simulink model "OffRoadMultibodyStage1_TireDamping_Cz20_20261101"  (R2026a)
settings: Solver=ode15s  StopTime=100  RelTol=2e-3  EnableMultiTasking=on
values from neighbouring files (symbols this model uses):
  goalX = goalPoseWorkflow(1)    [buildCustomPhysicalScenarioModel.m]    (also in correctCustomObstacle3Spawn.m; createScenarioIntegrationTestModel.m = goalPose(1); planAroundConfiguredObstacle.m = originalPath(end,1); restoreRoughTerrainWorkspace.m = goalXY(1))
  goalY = goalPoseWorkflow(2)    [buildCustomPhysicalScenarioModel.m]    (also in correctCustomObstacle3Spawn.m; createScenarioIntegrationTestModel.m = goalPose(2); planAroundConfiguredObstacle.m = originalPath(end,2); restoreRoughTerrainWorkspace.m = goalXY(2))
  obstacle3X = obs(3).centerXY(1)    [buildCustomPhysicalScenarioModel.m]    (also in correctCustomObstacle3Spawn.m = o3.centerXY(1); createScenarioIntegrationTestModel.m = obstacleXs(3); restoreRoughTerrainWorkspace.m = obstacleXs(3); runCustomObstacle5DelayedAblation32s.m = double(obs(3).centerXY(1)))
  obstacle3Y = obs(3).centerXY(2)    [buildCustomPhysicalScenarioModel.m]    (also in correctCustomObstacle3Spawn.m = o3.centerXY(2); createScenarioIntegrationTestModel.m = obstacleYs(3); restoreRoughTerrainWorkspace.m = obstacleYs(3); runCustomObstacle5DelayedAblation32s.m = double(obs(3).centerXY(2)))
  obstacleSpawnTime = [obstacleSpawnTime nan(1,4)]    [buildCustomPhysicalScenarioModel.m]    (also in correctCustomObstacle3Spawn.m = [[obs.spawnTime] nan(1,4)]; createScenarioIntegrationTestModel.m = [obs.spawnTime]; restoreRoughTerrainWorkspace.m = [obs.spawnTime]; runCustomObstacle5DelayedAblation32s.m = [[obs.spawnTime] nan(1,4)])
  obstacleXs = [obstacleXs nan(1,4)]    [buildCustomPhysicalScenarioModel.m]    (also in correctCustomObstacle3Spawn.m = [allCenters(:,1).' nan(1,4)]; createScenarioIntegrationTestModel.m = allCenters(:,1).'; onlineReplanFromPose.m = obstacleXs(valid); onlineReplanFromPoseGeometryAware.m = obstacleXs(valid))
  obstacleYs = [obstacleYs nan(1,4)]    [buildCustomPhysicalScenarioModel.m]    (also in correctCustomObstacle3Spawn.m = [allCenters(:,2).' nan(1,4)]; createScenarioIntegrationTestModel.m = allCenters(:,2).'; onlineReplanFromPose.m = obstacleYs(valid); onlineReplanFromPoseGeometryAware.m = obstacleYs(valid))
  originalPathPadded = [ ... (first row only)    [planAroundConfiguredObstacle.m]
  s = blockNames{k}    [inspectPhysicalScenarioModel.m]    (also in inspectSteeringControllerAndTransferFcn.m = strtrim(s); inspectSteeringJointSignalPath.m = valueToText(v); runCustomSolverProfiler40s.m = profileResult.summary)
  X = X(:)'    [launchElevationTerrainRoverViewer.m]    (also in launchElevationTerrainRoverViewerMultiDynamic.m; launchRoughTerrainScenarioEditor.m = double(evalin('base', 'X')); previewGeometryAwareObstaclePlanner.m = evalin('base','X'))
  Y = Y(:)    [launchElevationTerrainRoverViewer.m]    (also in launchElevationTerrainRoverViewerMultiDynamic.m; launchRoughTerrainScenarioEditor.m = double(evalin('base', 'Y')); previewGeometryAwareObstaclePlanner.m = evalin('base','Y'))
  Z = double(Z_multibody)    [inspectFailureLocation.m]    (also in launchElevationTerrainRoverViewer.m = ZGridSurface.'; launchElevationTerrainRoverViewerMultiDynamic.m = ZGridSurface.'; previewGeometryAwareObstaclePlanner.m = evalin('base','Z'))
libraries: nesl_utility x71, sm_lib x45, slpidlib x1
(part 1 of 2)
settings Model: Creator=sagar  LastModifiedBy=sagar
settings DebuggingCC: SubsystemReferenceDiagnosticForUnitTest=warning
settings SimscapeCC: SimscapeNominalValues="[{\"value\":\"1\",\"unit\":\"A\"},{\"value\":\"1\",\"unit\":\"bar\"},{\"value\":\"1\",\"unit\":\"cm^2\"},{\"value\":\"1\",\"unit\":\"cm^3/s\"},{\"value\":\"1\",\"unit\":\"kJ/kg\"},{\"value\":\"1\",\"unit\":\"kW\"},{\"value\":\"1\",\"unit\":\"l\"},{\"value\":\"1\",\"unit\":\"N\"},{\"value\":\"1\",\"unit\":\"N*m\"},{\"value\":\"1\",\"unit\":\"V\"}]"
settings ExplorerConfigSet: InternalSimMechanicsExplorerSettings=|
  | <ExplorerConfiguration>
  | 
  |   <canonicalview>default</canonicalview>
  | 
  |   <TilePanel>
  |     <TileInfo>
  |       <Tiles Columns="1" Count="1" Height="825" Rows="1" Width="1462">
  |         <Row Weight="1"/>
  |         <Column Weight="1"/>
  |         <Tile Height="1" Width="1" X="0" Y="0"/>
  |       </Tiles>
  |     </TileInfo>
  |     <SceneInfo>
  |       <SceneViewer>
  |         <IsThisViewStd>
  |           <IsStandardView>off</IsStandardView>
  |           <StandardViewName>Front</StandardViewName>
  |         </IsThisViewStd>
  |         <BGColor>
  |           <R>1</R>
  |           <G>1</G>
  |           <B>1</B>
  |           <A>1</A>
  |         </BGColor>
  |         <Camera>
  |           <DoPerspective>off</DoPerspective>
  |           <Position>
  |             <X>25</X>
  |             <Y>-125.54576462577884</Y>
  |             <Z>151.6388221817023</Z>
  |           </Position>
  |           <Center>
  |             <X>25</X>
  |             <Y>25</Y>
  |             <Z>1.0930575559234619</Z>
  |           </Center>
  |           <Up>
  |             <X>0</X>
  |             <Y>0.70710678118654757</Y>
  |             <Z>0.70710678118654757</Z>
  |           </Up>
  |           <XLim>20.406588216402103</XLim>
  |           <YLim>20.406588216402103</YLim>
  |           <ViewLimDist>0.01</ViewLimDist>
  |         </Camera>
  |       </SceneViewer>
  |     </SceneInfo>
  |   </TilePanel>
  | 
  |   <MechEditorPanel>
  |     <GfxPanelCameraMap/>
  |     <Cameras/>
  |     <VideoCreator>
  |       <IncludeTiles>All</IncludeTiles>
  |       <IncludeTime>on</IncludeTime>
  |       <IncludeWorldFrame>off</IncludeWorldFrame>
  |       <PlaybackSpeedRatio>1</PlaybackSpeedRatio>
  |       <FrameRate>30</FrameRate>
  |       <FrameSize>auto</FrameSize>
  |       <VideoFormat>UncompressedAVI</VideoFormat>
  |     </VideoCreator>
  |   </MechEditorPanel>
  | 
  |   <PlaybackSettings>
  |     <PlaybackSpeedFactor>16</PlaybackSpeedFactor>
  |   </PlaybackSettings>
  | 
  | </ExplorerConfiguration>

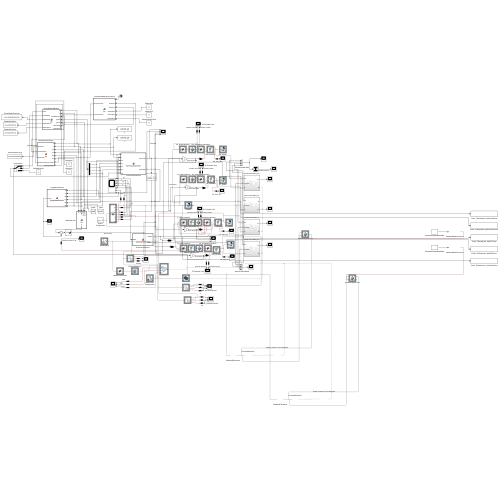
[thumbnail: Simulink's stored preview of the top-level diagram]
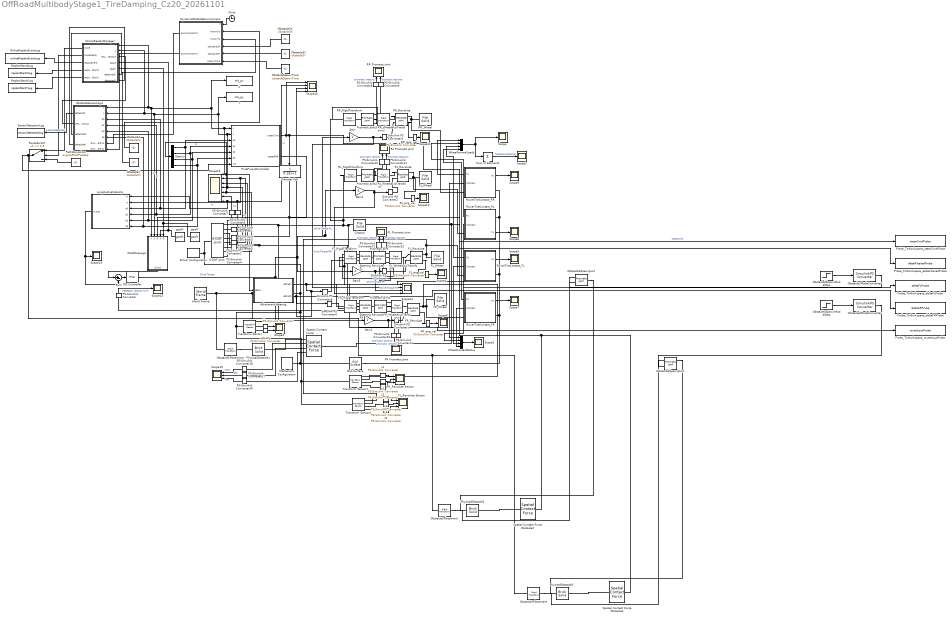
== system OffRoadMultibodyStage1_TireDamping_Cz20_20261101 ==
  6-DOF Joint : sm_lib/Joints/6-DOF Joint  JointMode=Normal  CompositeWrenchDir=FollowerOnBase  CompositeWrenchFrame=BaseFrame  SenseConstraintForce=off  SenseConstraintTorque=off  SenseTotalForce=off  SenseTotalTorque=off  PxPositionTargetSpecify=on  PxPositionTargetPriority=High  PxPositionTargetValue=4.53703703703703  PxPositionTargetValueUnits=m  PxVelocityTargetSpecify=off  PxVelocityTargetPriority=High  PxVelocityTargetValue=0  PxVelocityTargetValueUnits=m/s  PxEquilibriumPosition=0  PxEquilibriumPositionUnits=m  PxSpringStiffness=0  PxSpringStiffnessUnits=N/m  PxDampingCoefficient=0  PxDampingCoefficientUnits=N/(m/s)  PxLowerLimitSpecify=off  PxLowerLimitBound=-1  PxLowerLimitBoundUnits=m  PxLowerLimitStiffness=1e6  PxLowerLimitStiffnessUnits=N/m  PxLowerLimitDamping=1e3  PxLowerLimitDampingUnits=N/(m/s)  PxLowerLimitTransitionRegionWidth=1e-4  PxLowerLimitTransitionRegionWidthUnits=m  PxUpperLimitSpecify=off  PxUpperLimitBound=1  PxUpperLimitBoundUnits=m  PxUpperLimitStiffness=1e6  PxUpperLimitStiffnessUnits=N/m  PxUpperLimitDamping=1e3  PxUpperLimitDampingUnits=N/(m/s)  PxUpperLimitTransitionRegionWidth=1e-4  PxUpperLimitTransitionRegionWidthUnits=m  PxTorqueActuationMode=NoTorque  PxMotionActuationMode=ComputedMotion  PxSensePosition=on  PxSenseVelocity=on  PxSenseAcceleration=off  PxSenseTorqueForce=off  PxSenseLowerLimitTorqueForce=off  PxSenseUpperLimitTorqueForce=off  PyPositionTargetSpecify=on  PyPositionTargetPriority=High  PyPositionTargetValue=7.62345679012346  PyPositionTargetValueUnits=m  PyVelocityTargetSpecify=off  PyVelocityTargetPriority=High  PyVelocityTargetValue=0  PyVelocityTargetValueUnits=m/s  PyEquilibriumPosition=0  PyEquilibriumPositionUnits=m  PySpringStiffness=0  PySpringStiffnessUnits=N/m  PyDampingCoefficient=0  PyDampingCoefficientUnits=N/(m/s)  PyLowerLimitSpecify=off  PyLowerLimitBound=-1  PyLowerLimitBoundUnits=m  PyLowerLimitStiffness=1e6  PyLowerLimitStiffnessUnits=N/m  PyLowerLimitDamping=1e3  PyLowerLimitDampingUnits=N/(m/s)  PyLowerLimitTransitionRegionWidth=1e-4  PyLowerLimitTransitionRegionWidthUnits=m  PyUpperLimitSpecify=off  PyUpperLimitBound=1  PyUpperLimitBoundUnits=m  PyUpperLimitStiffness=1e6  PyUpperLimitStiffnessUnits=N/m  PyUpperLimitDamping=1e3  PyUpperLimitDampingUnits=N/(m/s)  PyUpperLimitTransitionRegionWidth=1e-4  PyUpperLimitTransitionRegionWidthUnits=m  PyTorqueActuationMode=NoTorque  PyMotionActuationMode=ComputedMotion  PySensePosition=on  PySenseVelocity=on  PySenseAcceleration=off  PySenseTorqueForce=off  PySenseLowerLimitTorqueForce=off  PySenseUpperLimitTorqueForce=off  PzPositionTargetSpecify=on  PzPositionTargetPriority=High  PzPositionTargetValue=0.15904942085294  PzPositionTargetValueUnits=m  PzVelocityTargetSpecify=off  PzVelocityTargetPriority=High  PzVelocityTargetValue=0  PzVelocityTargetValueUnits=m/s  PzEquilibriumPosition=0  PzEquilibriumPositionUnits=m  PzSpringStiffness=0  PzSpringStiffnessUnits=N/m  PzDampingCoefficient=0  PzDampingCoefficientUnits=N/(m/s)  PzLowerLimitSpecify=off  PzLowerLimitBound=-1  PzLowerLimitBoundUnits=m  PzLowerLimitStiffness=1e6  PzLowerLimitStiffnessUnits=N/m  PzLowerLimitDamping=1e3  PzLowerLimitDampingUnits=N/(m/s)  PzLowerLimitTransitionRegionWidth=1e-4  PzLowerLimitTransitionRegionWidthUnits=m  PzUpperLimitSpecify=off  PzUpperLimitBound=1  PzUpperLimitBoundUnits=m  PzUpperLimitStiffness=1e6  PzUpperLimitStiffnessUnits=N/m  PzUpperLimitDamping=1e3  PzUpperLimitDampingUnits=N/(m/s)  PzUpperLimitTransitionRegionWidth=1e-4  PzUpperLimitTransitionRegionWidthUnits=m  PzTorqueActuationMode=NoTorque  PzMotionActuationMode=ComputedMotion  PzSensePosition=on  PzSenseVelocity=off  PzSenseAcceleration=off  PzSenseTorqueForce=off  PzSenseLowerLimitTorqueForce=off  PzSenseUpperLimitTorqueForce=off  SphPositionTargetSpecify=on  SphPositionTargetPriority=High  SphPositionTargetRotationMethod=Quaternion  SphPositionTargetFollAlignAxisA=+X  SphPositionTargetBaseAlignAxisA=+Y  SphPositionTargetFollAlignAxisB=+Y  SphPositionTargetBaseAlignAxisB=+Z  SphPositionTargetRotationStandardAxis=+Z  SphPositionTargetRotationAngle=0  SphPositionTargetRotationAngleUnits=deg  SphPositionTargetRotationArbitraryAxis=[0 0 1]  SphPositionTargetRotationSequenceAxes=FollowerAxes  SphPositionTargetRotationSequence=XYX  SphPositionTargetRotationSequenceAngles=[0 0 0]  SphPositionTargetRotationSequenceAnglesUnits=deg  SphPositionTargetRotationMatrix=[1 0 0;0 1 0;0 0 1]  SphPositionTargetQuaternion=[0.923879532511287 0 0 0.38268343236509]  SphVelocityTargetSpecify=off  SphVelocityTargetPriority=High  SphVelocityTargetValue=[0 0 0]  SphVelocityTargetValueUnits=deg/s  SphVelocityTargetInFollowerFrame=on  SphEqPosRotationMethod=None  SphEqPosFollAlignAxisA=+X  SphEqPosBaseAlignAxisA=+Y  SphEqPosFollAlignAxisB=+Y  SphEqPosBaseAlignAxisB=+Z  SphEqPosRotationStandardAxis=+Z  SphEqPosRotationAngle=0  SphEqPosRotationAngleUnits=deg  SphEqPosRotationArbitraryAxis=[0 0 1]  SphEqPosRotationSequenceAxes=FollowerAxes  SphEqPosRotationSequence=XYX  SphEqPosRotationSequenceAngles=[0 0 0]  SphEqPosRotationSequenceAnglesUnits=deg  SphEqPosRotationMatrix=[1 0 0;0 1 0;0 0 1]  SphEqPosQuaternion=[1 0 0 0]  SphSpringStiffness=0  SphSpringStiffnessUnits=N*m/deg  SphDampingCoefficient=0  SphDampingCoefficientUnits=N*m/(deg/s)  SphLowerLimitSpecify=off  SphLowerLimitBound=15  SphLowerLimitBoundUnits=deg  SphLowerLimitStiffness=1e4  SphLowerLimitStiffnessUnits=N*m/deg  SphLowerLimitDamping=10  SphLowerLimitDampingUnits=N*m/(deg/s)  SphLowerLimitTransitionRegionWidth=0.1  SphLowerLimitTransitionRegionWidthUnits=deg  SphUpperLimitSpecify=off  SphUpperLimitBound=45  SphUpperLimitBoundUnits=deg  SphUpperLimitStiffness=1e4  SphUpperLimitStiffnessUnits=N*m/deg  SphUpperLimitDamping=10  SphUpperLimitDampingUnits=N*m/(deg/s)  SphUpperLimitTransitionRegionWidth=0.1  SphUpperLimitTransitionRegionWidthUnits=deg  SphTorqueActuationMode=NoTorque  SphActuateTorqueX=off  SphActuateTorqueY=off  SphActuateTorqueZ=off  SphActuateTorque=off  SphActuationFrame=BaseFrame  SphSensePosition=on  SphSenseVelocityX=off  SphSenseVelocityY=off  SphSenseVelocityZ=on  SphSenseVelocity=off  SphSenseAccelerationX=off  SphSenseAccelerationY=off  SphSenseAccelerationZ=off  SphSenseAcceleration=off  SphSenseLowerLimitTorqueMag=off  SphSenseUpperLimitTorqueMag=off  SphSensingFrame=BaseFrame
  AckermannSteering : MATLAB Function  TreatAsAtomicUnit=on
  Chassis : sm_lib/Body Elements/File Solid  ExtGeomFileName=C:\Users\sagar\OneDrive\Documents\AutonomousNavigationRoughTerrain\Buggy chassis.STL  UnitType=Custom  ExtGeomFileUnits=mm  StepReaderType=HEX  ExportConvexHullGeometry=on  InertiaType=Custom  BasedOnType=Mass  Density=1000  DensityUnits=kg/m^3  Mass=20  MassUnits=kg  CenterOfMass=[820 200 950]  CenterOfMassUnits=mm  MomentsOfInertia=[1 1 1]  MomentsOfInertiaUnits=kg*m^2  ProductsOfInertia=[0 0 0]  ProductsOfInertiaUnits=kg*m^2  GraphicType=FromGeometry  MarkerShape=Sphere  MarkerSize=10  GraphicVisPropType=SimpleVisualProperties  GraphicDiffuseColor=[0.6667 0 0]  GraphicOpacity=1  GraphicSpecularColor=[0.5 0.5 0.5 1.0]  GraphicAmbientColor=[0.15 0.15 0.15 1.0]  GraphicEmissiveColor=[0.0 0.0 0.0 1.0]  GraphicShininess=75  DoExposeReferenceFrame=off  SerializedFrames=|
      | <Frames>
      | 
      |   <Frame>
      |     <Id>Frame1</Id>
      |     <Value>
      |       <Name>Centre of mass</Name>
      |       <Origin>
      |         <Source>CenterOfMassFrame</Source>
      |         <FeatureName></FeatureName>
      |       </Origin>
      |       <PrimaryAxis>
      |         <DefinedDirection>+X</DefinedDirection>
      |         <Source>ReferenceFrame</Source>
      |         <SourceDirection>+Z</SourceDirection>
      |         <FeatureName></FeatureName>
      |       </PrimaryAxis>
      |       <SecondaryAxis>
      |         <DefinedDirection>+Y</DefinedDirection>
      |         <Source>ReferenceFrame</Source>
      |         <SourceDirection>+X</SourceDirection>
      |         <FeatureName></FeatureName>
      |       </SecondaryAxis>
      |     </Value>
      |   </Frame>
      | 
      | </Frames>
  Clock : Clock
  Demux : Demux
  DynamicObstacleEnvironment : MATLAB Function  TreatAsAtomicUnit=on
  FL Prismatic joint : Scope  NumInputPorts=2
      settings: ActiveDisplayYMinimum=-0.14201466642607241  ActiveDisplayYMaximum=0.45057200196499747  DataLoggingVariableName=ScopeData20
  FL_Revolute : sm_lib/Joints/Revolute Joint  JointMode=Normal  CompositeWrenchDir=FollowerOnBase  CompositeWrenchFrame=BaseFrame  SenseConstraintForce=off  SenseConstraintTorque=off  SenseTotalForce=off  SenseTotalTorque=off  PositionTargetSpecify=off  PositionTargetPriority=High  PositionTargetValue=0  PositionTargetValueUnits=deg  VelocityTargetSpecify=off  VelocityTargetPriority=High  VelocityTargetValue=0  VelocityTargetValueUnits=deg/s  EquilibriumPosition=0  EquilibriumPositionUnits=deg  SpringStiffness=0  SpringStiffnessUnits=N*m/deg  DampingCoefficient=0  DampingCoefficientUnits=N*m/(deg/s)  LowerLimitSpecify=off  LowerLimitBound=-90  LowerLimitBoundUnits=deg  LowerLimitStiffness=1e4  LowerLimitStiffnessUnits=N*m/deg  LowerLimitDamping=10  LowerLimitDampingUnits=N*m/(deg/s)  LowerLimitTransitionRegionWidth=0.1  LowerLimitTransitionRegionWidthUnits=deg  UpperLimitSpecify=off  UpperLimitBound=90  UpperLimitBoundUnits=deg  UpperLimitStiffness=1e4  UpperLimitStiffnessUnits=N*m/deg  UpperLimitDamping=10  UpperLimitDampingUnits=N*m/(deg/s)  UpperLimitTransitionRegionWidth=0.1  UpperLimitTransitionRegionWidthUnits=deg  TorqueActuationMode=InputTorque  MotionActuationMode=ComputedMotion  SensePosition=off  SenseVelocity=on  SenseAcceleration=off  SenseTorqueForce=off  SenseLowerLimitTorqueForce=off  SenseUpperLimitTorqueForce=off
  FL_Revolute Sensor : Scope  NumInputPorts=3
      settings: ActiveDisplayYMinimum=-1  ActiveDisplayYMaximum=1  DataLoggingVariableName=ScopeData24
  FL_RigidTransform : sm_lib/Frames and Transforms/Rigid Transform  RotationMethod=StandardAxis  FollAlignAxisA=+X  BaseAlignAxisA=+Y  FollAlignAxisB=+Y  BaseAlignAxisB=+Z  RotationStandardAxis=+X  RotationAngle=0  RotationAngleUnits=deg  RotationArbitraryAxis=[0 0 1]  RotationSequenceAxes=FollowerAxes  RotationSequence=XYX  RotationSequenceAngles=[0 0 0]  RotationSequenceAnglesUnits=deg  RotationMatrix=[1 0 0;0 1 0;0 0 1]  Quaternion=[1 0 0 0]  TranslationMethod=Cartesian  TranslationCartesianOffset=[625 460 -65]  TranslationCartesianOffsetUnits=mm  TranslationStandardAxis=+Z  TranslationStandardOffset=0  TranslationStandardOffsetUnits=m  TranslationROffset=0  TranslationROffsetUnits=m  TranslationThetaOffset=0  TranslationThetaOffsetUnits=deg  TranslationZOffset=0  TranslationZOffsetUnits=m
  FL_Wheel : sm_lib/Body Elements/File Solid  ExtGeomFileName=C:\Users\sagar\OneDrive\Documents\AutonomousNavigationRoughTerrain\RR_Wheel.STL  UnitType=Custom  ExtGeomFileUnits=mm  StepReaderType=HEX  ExportConvexHullGeometry=off  InertiaType=Custom  BasedOnType=Mass  Density=1000  DensityUnits=kg/m^3  Mass=1  MassUnits=kg  CenterOfMass=[35 76 76]  CenterOfMassUnits=mm  MomentsOfInertia=[0.00162 0.00289 0.00162]  MomentsOfInertiaUnits=kg*m^2  ProductsOfInertia=[0 0 0]  ProductsOfInertiaUnits=kg*m^2  GraphicType=FromGeometry  MarkerShape=Sphere  MarkerSize=10  GraphicVisPropType=SimpleVisualProperties  GraphicDiffuseColor=[0 0 0]  GraphicOpacity=1  GraphicSpecularColor=[0.5 0.5 0.5 1.0]  GraphicAmbientColor=[0.15 0.15 0.15 1.0]  GraphicEmissiveColor=[0.0 0.0 0.0 1.0]  GraphicShininess=75  DoExposeReferenceFrame=off  SerializedFrames=|
      | <Frames>
      | 
      |   <Frame>
      |     <Id>Frame1</Id>
      |     <Value>
      |       <Name>F1</Name>
      |       <Origin>
      |         <Source>CenterOfMassFrame</Source>
      |         <FeatureName></FeatureName>
      |       </Origin>
      |       <PrimaryAxis>
      |         <DefinedDirection>+Z</DefinedDirection>
      |         <Source>ReferenceFrame</Source>
      |         <SourceDirection>+X</SourceDirection>
      |         <FeatureName></FeatureName>
      |       </PrimaryAxis>
      |       <SecondaryAxis>
      |         <DefinedDirection>+X</DefinedDirection>
      |         <Source>ReferenceFrame</Source>
      |         <SourceDirection>-Z</SourceDirection>
      |         <FeatureName></FeatureName>
      |       </SecondaryAxis>
      |     </Value>
      |   </Frame>
      | 
      | </Frames>
  FL_WheelAxisTransform : sm_lib/Frames and Transforms/Rigid Transform  RotationMethod=StandardAxis  FollAlignAxisA=+X  BaseAlignAxisA=+Y  FollAlignAxisB=+Y  BaseAlignAxisB=+Z  RotationStandardAxis=+X  RotationAngle=90  RotationAngleUnits=deg  RotationArbitraryAxis=[0 0 1]  RotationSequenceAxes=FollowerAxes  RotationSequence=XYX  RotationSequenceAngles=[0 0 0]  RotationSequenceAnglesUnits=deg  RotationMatrix=[1 0 0;0 1 0;0 0 1]  Quaternion=[1 0 0 0]  TranslationMethod=Cartesian  TranslationCartesianOffset=[0 0 0]  TranslationCartesianOffsetUnits=m  TranslationStandardAxis=+Z  TranslationStandardOffset=0  TranslationStandardOffsetUnits=m  TranslationROffset=0  TranslationROffsetUnits=m  TranslationThetaOffset=0  TranslationThetaOffsetUnits=deg  TranslationZOffset=0  TranslationZOffsetUnits=m
  FL_ang_vel : nesl_utility/PS-Simulink Converter  PhysicalDomain=network_engine_domain  SubClassName=ps_output  LeftPortType=input  RightPortType=output  PseudoPeriodic=off  Frequencies=[]  VectorFormat=inherit  Unit=rad/s  AffineConversion=off
  FR Prismatic joint : Scope  NumInputPorts=2
      settings: ActiveDisplayYMinimum=-1  ActiveDisplayYMaximum=1  DataLoggingVariableName=ScopeData21
  FR_Revolute : sm_lib/Joints/Revolute Joint  JointMode=Normal  CompositeWrenchDir=FollowerOnBase  CompositeWrenchFrame=BaseFrame  SenseConstraintForce=off  SenseConstraintTorque=off  SenseTotalForce=off  SenseTotalTorque=off  PositionTargetSpecify=off  PositionTargetPriority=High  PositionTargetValue=0  PositionTargetValueUnits=deg  VelocityTargetSpecify=off  VelocityTargetPriority=High  VelocityTargetValue=0  VelocityTargetValueUnits=deg/s  EquilibriumPosition=0  EquilibriumPositionUnits=deg  SpringStiffness=0  SpringStiffnessUnits=N*m/deg  DampingCoefficient=0  DampingCoefficientUnits=N*m/(deg/s)  LowerLimitSpecify=off  LowerLimitBound=-90  LowerLimitBoundUnits=deg  LowerLimitStiffness=1e4  LowerLimitStiffnessUnits=N*m/deg  LowerLimitDamping=10  LowerLimitDampingUnits=N*m/(deg/s)  LowerLimitTransitionRegionWidth=0.1  LowerLimitTransitionRegionWidthUnits=deg  UpperLimitSpecify=off  UpperLimitBound=90  UpperLimitBoundUnits=deg  UpperLimitStiffness=1e4  UpperLimitStiffnessUnits=N*m/deg  UpperLimitDamping=10  UpperLimitDampingUnits=N*m/(deg/s)  UpperLimitTransitionRegionWidth=0.1  UpperLimitTransitionRegionWidthUnits=deg  TorqueActuationMode=InputTorque  MotionActuationMode=ComputedMotion  SensePosition=off  SenseVelocity=on  SenseAcceleration=off  SenseTorqueForce=off  SenseLowerLimitTorqueForce=off  SenseUpperLimitTorqueForce=off
  FR_Revolute Sensor : Scope  NumInputPorts=3
      settings: ActiveDisplayYMinimum=-1  ActiveDisplayYMaximum=1  DataLoggingVariableName=ScopeData23
  FR_RigidTransform : sm_lib/Frames and Transforms/Rigid Transform  RotationMethod=StandardAxis  FollAlignAxisA=+X  BaseAlignAxisA=+Y  FollAlignAxisB=+Y  BaseAlignAxisB=+Z  RotationStandardAxis=+X  RotationAngle=0  RotationAngleUnits=deg  RotationArbitraryAxis=[0 0 1]  RotationSequenceAxes=FollowerAxes  RotationSequence=XYX  RotationSequenceAngles=[0 0 0]  RotationSequenceAnglesUnits=deg  RotationMatrix=[1 0 0;0 1 0;0 0 1]  Quaternion=[1 0 0 0]  TranslationMethod=Cartesian  TranslationCartesianOffset=[625 -460 -65]  TranslationCartesianOffsetUnits=mm  TranslationStandardAxis=+Z  TranslationStandardOffset=0  TranslationStandardOffsetUnits=m  TranslationROffset=0  TranslationROffsetUnits=m  TranslationThetaOffset=0  TranslationThetaOffsetUnits=deg  TranslationZOffset=0  TranslationZOffsetUnits=m
  FR_Wheel : sm_lib/Body Elements/File Solid  ExtGeomFileName=C:\Users\sagar\OneDrive\Documents\AutonomousNavigationRoughTerrain\RR_Wheel.STL  UnitType=Custom  ExtGeomFileUnits=mm  StepReaderType=HEX  ExportConvexHullGeometry=off  InertiaType=Custom  BasedOnType=Mass  Density=1000  DensityUnits=kg/m^3  Mass=1  MassUnits=kg  CenterOfMass=[35 76 76]  CenterOfMassUnits=mm  MomentsOfInertia=[0.00162 0.00289 0.00162]  MomentsOfInertiaUnits=kg*m^2  ProductsOfInertia=[0 0 0]  ProductsOfInertiaUnits=kg*m^2  GraphicType=FromGeometry  MarkerShape=Sphere  MarkerSize=10  GraphicVisPropType=SimpleVisualProperties  GraphicDiffuseColor=[0 0 0]  GraphicOpacity=1  GraphicSpecularColor=[0.5 0.5 0.5 1.0]  GraphicAmbientColor=[0.15 0.15 0.15 1.0]  GraphicEmissiveColor=[0.0 0.0 0.0 1.0]  GraphicShininess=75  DoExposeReferenceFrame=off  SerializedFrames=|
      | <Frames>
      | 
      |   <Frame>
      |     <Id>Frame1</Id>
      |     <Value>
      |       <Name>F1</Name>
      |       <Origin>
      |         <Source>CenterOfMassFrame</Source>
      |         <FeatureName></FeatureName>
      |       </Origin>
      |       <PrimaryAxis>
      |         <DefinedDirection>+Z</DefinedDirection>
      |         <Source>ReferenceFrame</Source>
      |         <SourceDirection>+X</SourceDirection>
      |         <FeatureName></FeatureName>
      |       </PrimaryAxis>
      |       <SecondaryAxis>
      |         <DefinedDirection>+X</DefinedDirection>
      |         <Source>ReferenceFrame</Source>
      |         <SourceDirection>+Z</SourceDirection>
      |         <FeatureName></FeatureName>
      |       </SecondaryAxis>
      |     </Value>
      |   </Frame>
      | 
      | </Frames>
  FR_WheelAxisTransform : sm_lib/Frames and Transforms/Rigid Transform  RotationMethod=StandardAxis  FollAlignAxisA=+X  BaseAlignAxisA=+Y  FollAlignAxisB=+Y  BaseAlignAxisB=+Z  RotationStandardAxis=+X  RotationAngle=-90  RotationAngleUnits=deg  RotationArbitraryAxis=[0 0 1]  RotationSequenceAxes=FollowerAxes  RotationSequence=XYX  RotationSequenceAngles=[0 0 0]  RotationSequenceAnglesUnits=deg  RotationMatrix=[1 0 0;0 1 0;0 0 1]  Quaternion=[1 0 0 0]  TranslationMethod=Cartesian  TranslationCartesianOffset=[0 0 0]  TranslationCartesianOffsetUnits=m  TranslationStandardAxis=+Z  TranslationStandardOffset=0  TranslationStandardOffsetUnits=m  TranslationROffset=0  TranslationROffsetUnits=m  TranslationThetaOffset=0  TranslationThetaOffsetUnits=deg  TranslationZOffset=0  TranslationZOffsetUnits=m
  FR_ang_vel : nesl_utility/PS-Simulink Converter  PhysicalDomain=network_engine_domain  SubClassName=ps_output  LeftPortType=input  RightPortType=output  PseudoPeriodic=off  Frequencies=[]  VectorFormat=inherit  Unit=rad/s  AffineConversion=off
  Gain : Gain
  Gain1 : Gain  Gain=-1
  Gain2 : Gain
  Gain3 : Gain  Gain=-1
  GoalStopLogic : MATLAB Function  TreatAsAtomicUnit=on
  Grid Surface : sm_lib/Curves and Surfaces/Grid Surface  XGridVector=X_mb  XGridVectorUnits=m  YGridVector=Y_mb  YGridVectorUnits=m  ZHeights=Z_mb  ZHeightsUnits=m  GraphicType=FromGeometry  GraphicVisPropType=AdvancedVisualProperties  GraphicDiffuseColor=[0.5 0.5 0.5]  GraphicOpacity=1  GraphicSpecularColor=[0.5 0.5 0.5 1.0]  GraphicAmbientColor=[0.15 0.15 0.15 1.0]  GraphicEmissiveColor=[0.0 0.0 0.0 1.0]  GraphicShininess=75
  LongitudinalVelocity : MATLAB Function  TreatAsAtomicUnit=on
  Mechanism Configuration : sm_lib/Utilities/Mechanism Configuration  UniformGravity=Constant  GravityVector=[0 0 -9.81]  GravityVectorUnits=m/s^2  LinearizationDelta=0.001  JointModeTransitionNonlinearIterations=2
  Obstacle1Placement : sm_lib/Frames and Transforms/Rigid Transform  RotationMethod=None  FollAlignAxisA=+X  BaseAlignAxisA=+Y  FollAlignAxisB=+Y  BaseAlignAxisB=+Z  RotationStandardAxis=+Z  RotationAngle=0  RotationAngleUnits=deg  RotationArbitraryAxis=[0 0 1]  RotationSequenceAxes=FollowerAxes  RotationSequence=XYX  RotationSequenceAngles=[0 0 0]  RotationSequenceAnglesUnits=deg  RotationMatrix=[1 0 0;0 1 0;0 0 1]  Quaternion=[1 0 0 0]  TranslationMethod=Cartesian  TranslationCartesianOffset=[5.77160493827 17.3148148148 1.72073998136]  TranslationCartesianOffsetUnits=m  TranslationStandardAxis=+Z  TranslationStandardOffset=0  TranslationStandardOffsetUnits=m  TranslationROffset=0  TranslationROffsetUnits=m  TranslationThetaOffset=0  TranslationThetaOffsetUnits=deg  TranslationZOffset=0  TranslationZOffsetUnits=m
  Obstacle2ModeConverter : nesl_utility/Simulink-PS Converter  PhysicalDomain=network_engine_domain  SubClassName=ps_input  LeftPortType=input  RightPortType=output  PseudoPeriodic=off  Frequencies=[]  NoiseDistribution=none  NoiseParameters=[]  Unit=1  AffineConversion=off  FilteringAndDerivatives=provide  SimscapeFilterOrder=1  InputFilterTimeConstant=0.001  UdotUserProvided=0
  Obstacle2Placement : sm_lib/Frames and Transforms/Rigid Transform  RotationMethod=None  FollAlignAxisA=+X  BaseAlignAxisA=+Y  FollAlignAxisB=+Y  BaseAlignAxisB=+Z  RotationStandardAxis=+Z  RotationAngle=0  RotationAngleUnits=deg  RotationArbitraryAxis=[0 0 1]  RotationSequenceAxes=FollowerAxes  RotationSequence=XYX  RotationSequenceAngles=[0 0 0]  RotationSequenceAnglesUnits=deg  RotationMatrix=[1 0 0;0 1 0;0 0 1]  Quaternion=[1 0 0 0]  TranslationMethod=Cartesian  TranslationCartesianOffset=[27.1913580247 18.8580246914 1.11734769361]  TranslationCartesianOffsetUnits=m  TranslationStandardAxis=+Z  TranslationStandardOffset=0  TranslationStandardOffsetUnits=m  TranslationROffset=0  TranslationROffsetUnits=m  TranslationThetaOffset=0  TranslationThetaOffsetUnits=deg  TranslationZOffset=0  TranslationZOffsetUnits=m
  Obstacle2SpawnJoint : sm_lib/Joints/Prismatic Joint  JointMode=ProvidedByInput  CompositeWrenchDir=FollowerOnBase  CompositeWrenchFrame=BaseFrame  SenseConstraintForce=off  SenseConstraintTorque=off  SenseTotalForce=off  SenseTotalTorque=off  PositionTargetSpecify=on  PositionTargetPriority=High  PositionTargetValue=0  PositionTargetValueUnits=m  VelocityTargetSpecify=off  VelocityTargetPriority=High  VelocityTargetValue=0  VelocityTargetValueUnits=m/s  EquilibriumPosition=0  EquilibriumPositionUnits=m  SpringStiffness=4000  SpringStiffnessUnits=N/m  DampingCoefficient=300  DampingCoefficientUnits=N/(m/s)  LowerLimitSpecify=off  LowerLimitBound=-1  LowerLimitBoundUnits=m  LowerLimitStiffness=1e6  LowerLimitStiffnessUnits=N/m  LowerLimitDamping=1e3  LowerLimitDampingUnits=N/(m/s)  LowerLimitTransitionRegionWidth=1e-4  LowerLimitTransitionRegionWidthUnits=m  UpperLimitSpecify=on  UpperLimitBound=0  UpperLimitBoundUnits=m  UpperLimitStiffness=1e5  UpperLimitStiffnessUnits=N/m  UpperLimitDamping=1500  UpperLimitDampingUnits=N/(m/s)  UpperLimitTransitionRegionWidth=0.005  UpperLimitTransitionRegionWidthUnits=m  TorqueActuationMode=NoTorque  MotionActuationMode=ComputedMotion  SensePosition=off  SenseVelocity=off  SenseAcceleration=off  SenseTorqueForce=off  SenseLowerLimitTorqueForce=off  SenseUpperLimitTorqueForce=off
  Obstacle2SpawnModeStep : Step  Time=0  InitialValue=1  SampleTime=0
  Obstacle3ModeConverter : nesl_utility/Simulink-PS Converter  PhysicalDomain=network_engine_domain  SubClassName=ps_input  LeftPortType=input  RightPortType=output  PseudoPeriodic=off  Frequencies=[]  NoiseDistribution=none  NoiseParameters=[]  Unit=1  AffineConversion=off  FilteringAndDerivatives=provide  SimscapeFilterOrder=1  InputFilterTimeConstant=0.001  UdotUserProvided=0
  Obstacle3Placement : sm_lib/Frames and Transforms/Rigid Transform  RotationMethod=None  FollAlignAxisA=+X  BaseAlignAxisA=+Y  FollAlignAxisB=+Y  BaseAlignAxisB=+Z  RotationStandardAxis=+Z  RotationAngle=0  RotationAngleUnits=deg  RotationArbitraryAxis=[0 0 1]  RotationSequenceAxes=FollowerAxes  RotationSequence=XYX  RotationSequenceAngles=[0 0 0]  RotationSequenceAnglesUnits=deg  RotationMatrix=[1 0 0;0 1 0;0 0 1]  Quaternion=[1 0 0 0]  TranslationMethod=Cartesian  TranslationCartesianOffset=[27.9938271605 27.0061728395 2.26509595869]  TranslationCartesianOffsetUnits=m  TranslationStandardAxis=+Z  TranslationStandardOffset=0  TranslationStandardOffsetUnits=m  TranslationROffset=0  TranslationROffsetUnits=m  TranslationThetaOffset=0  TranslationThetaOffsetUnits=deg  TranslationZOffset=0  TranslationZOffsetUnits=m
  Obstacle3SpawnJoint : sm_lib/Joints/Prismatic Joint  JointMode=ProvidedByInput  CompositeWrenchDir=FollowerOnBase  CompositeWrenchFrame=BaseFrame  SenseConstraintForce=off  SenseConstraintTorque=off  SenseTotalForce=off  SenseTotalTorque=off  PositionTargetSpecify=on  PositionTargetPriority=High  PositionTargetValue=-4.34068313022  PositionTargetValueUnits=m  VelocityTargetSpecify=off  VelocityTargetPriority=High  VelocityTargetValue=0  VelocityTargetValueUnits=m/s  EquilibriumPosition=9.81  EquilibriumPositionUnits=m  SpringStiffness=10  SpringStiffnessUnits=N/m  DampingCoefficient=20  DampingCoefficientUnits=N/(m/s)  LowerLimitSpecify=off  LowerLimitBound=-1  LowerLimitBoundUnits=m  LowerLimitStiffness=1e6  LowerLimitStiffnessUnits=N/m  LowerLimitDamping=1e3  LowerLimitDampingUnits=N/(m/s)  LowerLimitTransitionRegionWidth=1e-4  LowerLimitTransitionRegionWidthUnits=m  UpperLimitSpecify=on  UpperLimitBound=0  UpperLimitBoundUnits=m  UpperLimitStiffness=1e5  UpperLimitStiffnessUnits=N/m  UpperLimitDamping=1500  UpperLimitDampingUnits=N/(m/s)  UpperLimitTransitionRegionWidth=0.005  UpperLimitTransitionRegionWidthUnits=m  TorqueActuationMode=NoTorque  MotionActuationMode=ComputedMotion  SensePosition=off  SenseVelocity=off  SenseAcceleration=off  SenseTorqueForce=off  SenseLowerLimitTorqueForce=off  SenseUpperLimitTorqueForce=on
  Obstacle3SpawnModeStep : Step  Time=7  InitialValue=1  FinalValue=0  SampleTime=0
  Obstacle3X : Constant  Value=obstacle3X
  Obstacle3Y : Constant  Value=obstacle3Y
  ObstacleSensorLogic : MATLAB Function  TreatAsAtomicUnit=on
  ObstacleSpawnTime : Constant  Value=obstacleSpawnTime
  ObstacleX : Constant  Value=obstacleXs
  ObstacleY : Constant  Value=obstacleYs
  OnlineReplanEventLog : ToWorkspace  VariableName=onlineReplanEventLog  SaveFormat=Timeseries  SampleTime=-1
  OnlineReplanManager : MATLAB Function  TreatAsAtomicUnit=on
  PID Controller : slpidlib/PID Controller  Controller=PI  Form=Parallel  TimeDomain=Continuous-time  UseExternalTs=off  SampleTime=-1  IntegratorMethod=Forward Euler  FilterMethod=Forward Euler  ControllerParametersSource=internal  P=1  I=0.3  UseKiTs=off  D=0  UseExternalDerivativeSource=off  N=100  UseFilter=on  TunerSelectOption=Transfer Function Based (PID Tuner App)  InitialConditionSource=internal  InitialConditionForIntegrator=0  InitialConditionForFilter=0  DifferentiatorICPrevScaledInput=0  ExternalReset=none  TrackingMode=off  Kt=1  LimitOutput=on  SatLimitsSource=internal  UpperSaturationLimit=3  LowerSaturationLimit=-3  LinearizeAsGain=on  AntiWindupMode=back-calculation  Kb=1  LimitIntegrator=off  UpperIntegratorSaturationLimit=inf  LowerIntegratorSaturationLimit=-inf  POutMin=[]  POutMax=[]  IOutMin=[]  IOutMax=[]  DOutMin=[]  DOutMax=[]  NOutMin=[]  NOutMax=[]  SumOutMin=[]  SumOutMax=[]  SaturationOutMin=[]  SaturationOutMax=[]  PParamMin=[]  PParamMax=[]  IParamMin=[]  IParamMax=[]  DParamMin=[]  DParamMax=[]  NParamMin=[]  NParamMax=[]  KbParamMin=[]  KbParamMax=[]  KtParamMin=[]  KtParamMax=[]  KbOutMin=[]  KbOutMax=[]  KtOutMin=[]  KtOutMax=[]  IntegratorOutMin=[]  IntegratorOutMax=[]  FilterOutMin=[]  FilterOutMax=[]  SumI1OutMin=[]  SumI1OutMax=[]  SumI2OutMin=[]  SumI2OutMax=[]  SumI3OutMin=[]  SumI3OutMax=[]  SumI4OutMin=[]  SumI4OutMax=[]  SumDOutMin=[]  SumDOutMax=[]  DifferentiatorOutMin=[]  DifferentiatorOutMax=[]  FilterDiffOutCoefMin=[]  FilterDiffOutCoefMax=[]  ReciprocalOutMin=[]  ReciprocalOutMax=[]  SumDenOutMin=[]  SumDenOutMax=[]  SumNumOutMin=[]  SumNumOutMax=[]  DivideOutMin=[]  DivideOutMax=[]  UdiffTsProdOutMin=[]  UdiffTsProdOutMax=[]  NTsProdOutMin=[]  NTsProdOutMax=[]  UintegralTsProdOutMin=[]  UintegralTsProdOutMax=[]  UngainTsProdOutMin=[]  UngainTsProdOutMax=[]  ClampingZeroOutDataTypeStr=Inherit: Inherit via back propagation  ClampingZeroOutMin=[]  ClampingZeroOutMax=[]  FilterDenConstantOutDataTypeStr=Inherit: Inherit via back propagation  FilterDenConstantOutMin=[]  FilterDenConstantOutMax=[]  PCopyOutDataTypeStr=Inherit: Inherit via back propagation  PCopyOutMin=[]  PCopyOutMax=[]  NCopyOutDataTypeStr=Inherit: Inherit via back propagation  NCopyOutMin=[]  NCopyOutMax=[]  IntegratorContinuousStateAttributes=''  IntegratorStateMustResolveToSignalObject=off  IntegratorRTWStateStorageClass=Auto  FilterContinuousStateAttributes=''  FilterStateMustResolveToSignalObject=off  FilterRTWStateStorageClass=Auto  ParallelPVariant=InternalParameters  IdealPVariant=Disabled  IVariant=InternalParameters  DVariant=Disabled  IntegratorVariant=Continuous  SatVariant=Enabled  AWVariant=BackCalculation  PCopyVariant=Disabled  TRVariant=Disabled  FdbkBlocksVariant=Forward  IdealPFdbkVariant=Disabled  SatFdbkVariant=Disabled  DerivativeFilterVariant=Disabled  NVariant=Disabled  NCopyVariant=Disabled_SignalSpec  FilterICVariant=Disabled  IntegratorICVariant=InternalICs  ExternalResetVariant=Disabled  TRSumVariant=Passthrough  SumFdbkVariant=Disabled  SumVariant=Sum_PI  TsampFilterVariant=InternalTs  TsampNgainVariant=Passthrough  TsampIntegralVariant=Disabled_SignalSpec  ExternalSaturationOutDataTypeStr=Inherit: Same as second input  DerivativeSourceVariant=Disabled  PreIntVariant=InternalPreInt
  PS-Simulink Converter{,1..18} (19 alike) : nesl_utility/PS-Simulink Converter  PhysicalDomain=network_engine_domain  SubClassName=ps_output  LeftPortType=input  RightPortType=output  PseudoPeriodic=off  Frequencies=[]  VectorFormat=inherit  Unit=inherit  AffineConversion=off
  PathWaypoints : Constant  Value=originalPathPadded
  PhysicalObstacle1 : sm_lib/Body Elements/Brick Solid  BrickDimensions=[5 5 2]  BrickDimensionsUnits=m  ExportEntireGeometry=on  InertiaType=CalculateFromGeometry  BasedOnType=Density  Density=1000  DensityUnits=kg/m^3  Mass=1  MassUnits=kg  CenterOfMass=[0 0 0]  CenterOfMassUnits=m  MomentsOfInertia=[1 1 1]  MomentsOfInertiaUnits=kg*m^2  ProductsOfInertia=[0 0 0]  ProductsOfInertiaUnits=kg*m^2  GraphicType=FromGeometry  MarkerShape=Sphere  MarkerSize=10  GraphicVisPropType=SimpleVisualProperties  GraphicDiffuseColor=[1 1 0]  GraphicOpacity=1  GraphicSpecularColor=[0.5 0.5 0.5 1.0]  GraphicAmbientColor=[0.15 0.15 0.15 1.0]  GraphicEmissiveColor=[0.0 0.0 0.0 1.0]  GraphicShininess=75  DoExposeReferenceFrame=on  SerializedFrames=<Frames/>
  PhysicalObstacle2 : sm_lib/Body Elements/Brick Solid  BrickDimensions=[17 4 2]  BrickDimensionsUnits=m  ExportEntireGeometry=on  InertiaType=CalculateFromGeometry  BasedOnType=Mass  Density=1000  DensityUnits=kg/m^3  Mass=25  MassUnits=kg  CenterOfMass=[0 0 0]  CenterOfMassUnits=m  MomentsOfInertia=[1 1 1]  MomentsOfInertiaUnits=kg*m^2  ProductsOfInertia=[0 0 0]  ProductsOfInertiaUnits=kg*m^2  GraphicType=FromGeometry  MarkerShape=Sphere  MarkerSize=10  GraphicVisPropType=SimpleVisualProperties  GraphicDiffuseColor=[1 1 0]  GraphicOpacity=1  GraphicSpecularColor=[0.5 0.5 0.5 1.0]  GraphicAmbientColor=[0.15 0.15 0.15 1.0]  GraphicEmissiveColor=[0.0 0.0 0.0 1.0]  GraphicShininess=75  DoExposeReferenceFrame=on  SerializedFrames=<Frames/>
  PhysicalObstacle3 : sm_lib/Body Elements/Brick Solid  BrickDimensions=[4 8 4]  BrickDimensionsUnits=m  ExportEntireGeometry=on  InertiaType=CalculateFromGeometry  BasedOnType=Mass  Density=1000  DensityUnits=kg/m^3  Mass=10  MassUnits=kg  CenterOfMass=[0 0 0]  CenterOfMassUnits=m  MomentsOfInertia=[1 1 1]  MomentsOfInertiaUnits=kg*m^2  ProductsOfInertia=[0 0 0]  ProductsOfInertiaUnits=kg*m^2  GraphicType=FromGeometry  MarkerShape=Sphere  MarkerSize=10  GraphicVisPropType=SimpleVisualProperties  GraphicDiffuseColor=[1 1 0]  GraphicOpacity=1  GraphicSpecularColor=[0.5 0.5 0.5 1.0]  GraphicAmbientColor=[0.15 0.15 0.15 1.0]  GraphicEmissiveColor=[0.0 0.0 0.0 1.0]  GraphicShininess=75  DoExposeReferenceFrame=on  SerializedFrames=<Frames/>
  Prismatic Joint{,1..3} (4 alike) : sm_lib/Joints/Prismatic Joint  JointMode=Normal  CompositeWrenchDir=FollowerOnBase  CompositeWrenchFrame=BaseFrame  SenseConstraintForce=off  SenseConstraintTorque=off  SenseTotalForce=off  SenseTotalTorque=off  PositionTargetSpecify=off  PositionTargetPriority=High  PositionTargetValue=0  PositionTargetValueUnits=m  VelocityTargetSpecify=off  VelocityTargetPriority=High  VelocityTargetValue=0  VelocityTargetValueUnits=m/s  EquilibriumPosition=0  EquilibriumPositionUnits=m  SpringStiffness=4000  SpringStiffnessUnits=N/m  DampingCoefficient=300  DampingCoefficientUnits=N/(m/s)  LowerLimitSpecify=off  LowerLimitBound=-1  LowerLimitBoundUnits=m  LowerLimitStiffness=1e6  LowerLimitStiffnessUnits=N/m  LowerLimitDamping=1e3  LowerLimitDampingUnits=N/(m/s)  LowerLimitTransitionRegionWidth=1e-4  LowerLimitTransitionRegionWidthUnits=m  UpperLimitSpecify=off  UpperLimitBound=1  UpperLimitBoundUnits=m  UpperLimitStiffness=1e6  UpperLimitStiffnessUnits=N/m  UpperLimitDamping=1e3  UpperLimitDampingUnits=N/(m/s)  UpperLimitTransitionRegionWidth=1e-4  UpperLimitTransitionRegionWidthUnits=m  TorqueActuationMode=NoTorque  MotionActuationMode=ComputedMotion  SensePosition=on  SenseVelocity=on  SenseAcceleration=off  SenseTorqueForce=off  SenseLowerLimitTorqueForce=off  SenseUpperLimitTorqueForce=off
  Probe_ToWorkspace_deltaFLProbe : ToWorkspace  VariableName=deltaFLProbe  SaveFormat=Timeseries  SampleTime=-1
  Probe_ToWorkspace_deltaFRProbe : ToWorkspace  VariableName=deltaFRProbe  SaveFormat=Timeseries  SampleTime=-1
  Probe_ToWorkspace_deltaFilteredProbe : ToWorkspace  VariableName=deltaFilteredProbe  SaveFormat=Timeseries  SampleTime=-1
  Probe_ToWorkspace_routeInputProbe : ToWorkspace  VariableName=routeInputProbe  SaveFormat=Timeseries  SampleTime=-1
  Probe_ToWorkspace_steerCmdProbe : ToWorkspace  VariableName=steerCmdProbe  SaveFormat=Timeseries  SampleTime=-1
  PurePursuitController : MATLAB Function  TreatAsAtomicUnit=on
  RL Prismatic joint : Scope  NumInputPorts=2
      settings: ActiveDisplayYMinimum=-1  ActiveDisplayYMaximum=1  DataLoggingVariableName=ScopeData19
  RL_Revolute : sm_lib/Joints/Revolute Joint  JointMode=Normal  CompositeWrenchDir=FollowerOnBase  CompositeWrenchFrame=BaseFrame  SenseConstraintForce=off  SenseConstraintTorque=off  SenseTotalForce=off  SenseTotalTorque=off  PositionTargetSpecify=off  PositionTargetPriority=High  PositionTargetValue=0  PositionTargetValueUnits=deg  VelocityTargetSpecify=off  VelocityTargetPriority=High  VelocityTargetValue=0  VelocityTargetValueUnits=deg/s  EquilibriumPosition=0  EquilibriumPositionUnits=deg  SpringStiffness=0  SpringStiffnessUnits=N*m/deg  DampingCoefficient=0  DampingCoefficientUnits=N*m/(deg/s)  LowerLimitSpecify=off  LowerLimitBound=-90  LowerLimitBoundUnits=deg  LowerLimitStiffness=1e4  LowerLimitStiffnessUnits=N*m/deg  LowerLimitDamping=10  LowerLimitDampingUnits=N*m/(deg/s)  LowerLimitTransitionRegionWidth=0.1  LowerLimitTransitionRegionWidthUnits=deg  UpperLimitSpecify=off  UpperLimitBound=90  UpperLimitBoundUnits=deg  UpperLimitStiffness=1e4  UpperLimitStiffnessUnits=N*m/deg  UpperLimitDamping=10  UpperLimitDampingUnits=N*m/(deg/s)  UpperLimitTransitionRegionWidth=0.1  UpperLimitTransitionRegionWidthUnits=deg  TorqueActuationMode=InputTorque  MotionActuationMode=ComputedMotion  SensePosition=off  SenseVelocity=on  SenseAcceleration=off  SenseTorqueForce=off  SenseLowerLimitTorqueForce=off  SenseUpperLimitTorqueForce=off
  RL_RigidTransform : sm_lib/Frames and Transforms/Rigid Transform  RotationMethod=StandardAxis  FollAlignAxisA=+X  BaseAlignAxisA=+Y  FollAlignAxisB=+Y  BaseAlignAxisB=+Z  RotationStandardAxis=+X  RotationAngle=0  RotationAngleUnits=deg  RotationArbitraryAxis=[0 0 1]  RotationSequenceAxes=FollowerAxes  RotationSequence=XYX  RotationSequenceAngles=[0 0 0]  RotationSequenceAnglesUnits=deg  RotationMatrix=[1 0 0;0 1 0;0 0 1]  Quaternion=[1 0 0 0]  TranslationMethod=Cartesian  TranslationCartesianOffset=[-490 445 -40]  TranslationCartesianOffsetUnits=mm  TranslationStandardAxis=+Z  TranslationStandardOffset=0  TranslationStandardOffsetUnits=m  TranslationROffset=0  TranslationROffsetUnits=m  TranslationThetaOffset=0  TranslationThetaOffsetUnits=deg  TranslationZOffset=0  TranslationZOffsetUnits=m
  RL_Wheel : sm_lib/Body Elements/File Solid  ExtGeomFileName=C:\Users\sagar\OneDrive\Documents\AutonomousNavigationRoughTerrain\RR_Wheel.STL  UnitType=Custom  ExtGeomFileUnits=mm  StepReaderType=HEX  ExportConvexHullGeometry=off  InertiaType=Custom  BasedOnType=Mass  Density=1000  DensityUnits=kg/m^3  Mass=1  MassUnits=kg  CenterOfMass=[35 76 76]  CenterOfMassUnits=mm  MomentsOfInertia=[0.00162 0.00289 0.00162]  MomentsOfInertiaUnits=kg*m^2  ProductsOfInertia=[0 0 0]  ProductsOfInertiaUnits=kg*m^2  GraphicType=FromGeometry  MarkerShape=Sphere  MarkerSize=10  GraphicVisPropType=SimpleVisualProperties  GraphicDiffuseColor=[0 0 0]  GraphicOpacity=1  GraphicSpecularColor=[0.5 0.5 0.5 1.0]  GraphicAmbientColor=[0.15 0.15 0.15 1.0]  GraphicEmissiveColor=[0.0 0.0 0.0 1.0]  GraphicShininess=75  DoExposeReferenceFrame=off  SerializedFrames=|
      | <Frames>
      | 
      |   <Frame>
      |     <Id>Frame1</Id>
      |     <Value>
      |       <Name>F1</Name>
      |       <Origin>
      |         <Source>CenterOfMassFrame</Source>
      |         <FeatureName></FeatureName>
      |       </Origin>
      |       <PrimaryAxis>
      |         <DefinedDirection>+Y</DefinedDirection>
      |         <Source>ReferenceFrame</Source>
      |         <SourceDirection>+Y</SourceDirection>
      |         <FeatureName></FeatureName>
      |       </PrimaryAxis>
      |       <SecondaryAxis>
      |         <DefinedDirection>+Z</DefinedDirection>
      |         <Source>ReferenceFrame</Source>
      |         <SourceDirection>+X</SourceDirection>
      |         <FeatureName></FeatureName>
      |       </SecondaryAxis>
      |     </Value>
      |   </Frame>
      | 
      | </Frames>
  RL_WheelAxisTransform : sm_lib/Frames and Transforms/Rigid Transform  RotationMethod=StandardAxis  FollAlignAxisA=+X  BaseAlignAxisA=+Y  FollAlignAxisB=+Y  BaseAlignAxisB=+Z  RotationStandardAxis=+X  RotationAngle=90  RotationAngleUnits=deg  RotationArbitraryAxis=[0 0 1]  RotationSequenceAxes=FollowerAxes  RotationSequence=XYX  RotationSequenceAngles=[0 0 0]  RotationSequenceAnglesUnits=deg  RotationMatrix=[1 0 0;0 1 0;0 0 1]  Quaternion=[1 0 0 0]  TranslationMethod=Cartesian  TranslationCartesianOffset=[0 0 0]  TranslationCartesianOffsetUnits=m  TranslationStandardAxis=+Z  TranslationStandardOffset=0  TranslationStandardOffsetUnits=m  TranslationROffset=0  TranslationROffsetUnits=m  TranslationThetaOffset=0  TranslationThetaOffsetUnits=deg  TranslationZOffset=0  TranslationZOffsetUnits=m
  RL_ang_vel : nesl_utility/PS-Simulink Converter  PhysicalDomain=network_engine_domain  SubClassName=ps_output  LeftPortType=input  RightPortType=output  PseudoPeriodic=off  Frequencies=[]  VectorFormat=inherit  Unit=rad/s  AffineConversion=off
  RR Prismatic joint : Scope  NumInputPorts=2
      settings: ActiveDisplayYMinimum=-0.21948307705397219  ActiveDisplayYMaximum=0.83635090870341677  DataLoggingVariableName=ScopeData18
  RR_Revolute : sm_lib/Joints/Revolute Joint  JointMode=Normal  CompositeWrenchDir=FollowerOnBase  CompositeWrenchFrame=BaseFrame  SenseConstraintForce=off  SenseConstraintTorque=off  SenseTotalForce=off  SenseTotalTorque=off  PositionTargetSpecify=off  PositionTargetPriority=High  PositionTargetValue=0  PositionTargetValueUnits=deg  VelocityTargetSpecify=off  VelocityTargetPriority=High  VelocityTargetValue=0  VelocityTargetValueUnits=deg/s  EquilibriumPosition=0  EquilibriumPositionUnits=deg  SpringStiffness=0  SpringStiffnessUnits=N*m/deg  DampingCoefficient=0  DampingCoefficientUnits=N*m/(deg/s)  LowerLimitSpecify=off  LowerLimitBound=-90  LowerLimitBoundUnits=deg  LowerLimitStiffness=1e4  LowerLimitStiffnessUnits=N*m/deg  LowerLimitDamping=10  LowerLimitDampingUnits=N*m/(deg/s)  LowerLimitTransitionRegionWidth=0.1  LowerLimitTransitionRegionWidthUnits=deg  UpperLimitSpecify=off  UpperLimitBound=90  UpperLimitBoundUnits=deg  UpperLimitStiffness=1e4  UpperLimitStiffnessUnits=N*m/deg  UpperLimitDamping=10  UpperLimitDampingUnits=N*m/(deg/s)  UpperLimitTransitionRegionWidth=0.1  UpperLimitTransitionRegionWidthUnits=deg  TorqueActuationMode=InputTorque  MotionActuationMode=ComputedMotion  SensePosition=off  SenseVelocity=on  SenseAcceleration=off  SenseTorqueForce=off  SenseLowerLimitTorqueForce=off  SenseUpperLimitTorqueForce=off
  RR_RigidTransform : sm_lib/Frames and Transforms/Rigid Transform  RotationMethod=StandardAxis  FollAlignAxisA=+X  BaseAlignAxisA=+Y  FollAlignAxisB=+Y  BaseAlignAxisB=+Z  RotationStandardAxis=+X  RotationAngle=0  RotationAngleUnits=deg  RotationArbitraryAxis=[0 0 1]  RotationSequenceAxes=FollowerAxes  RotationSequence=XYX  RotationSequenceAngles=[0 0 0]  RotationSequenceAnglesUnits=deg  RotationMatrix=[1 0 0;0 1 0;0 0 1]  Quaternion=[1 0 0 0]  TranslationMethod=Cartesian  TranslationCartesianOffset=[-490 -445 -40]  TranslationCartesianOffsetUnits=mm  TranslationStandardAxis=+Z  TranslationStandardOffset=0  TranslationStandardOffsetUnits=m  TranslationROffset=0  TranslationROffsetUnits=m  TranslationThetaOffset=0  TranslationThetaOffsetUnits=deg  TranslationZOffset=0  TranslationZOffsetUnits=m
  RR_Wheel : sm_lib/Body Elements/File Solid  ExtGeomFileName=C:\Users\sagar\OneDrive\Documents\AutonomousNavigationRoughTerrain\RR_Wheel.STL  UnitType=Custom  ExtGeomFileUnits=mm  StepReaderType=HEX  ExportConvexHullGeometry=off  InertiaType=Custom  BasedOnType=Mass  Density=1000  DensityUnits=kg/m^3  Mass=1  MassUnits=kg  CenterOfMass=[35 76 76]  CenterOfMassUnits=mm  MomentsOfInertia=[0.00162 0.00289 0.00162]  MomentsOfInertiaUnits=kg*m^2  ProductsOfInertia=[0 0 0]  ProductsOfInertiaUnits=kg*m^2  GraphicType=FromGeometry  MarkerShape=Sphere  MarkerSize=10  GraphicVisPropType=SimpleVisualProperties  GraphicDiffuseColor=[0 0 0]  GraphicOpacity=1  GraphicSpecularColor=[0.5 0.5 0.5 1.0]  GraphicAmbientColor=[0.15 0.15 0.15 1.0]  GraphicEmissiveColor=[0.0 0.0 0.0 1.0]  GraphicShininess=75  DoExposeReferenceFrame=off  SerializedFrames=|
      | <Frames>
      | 
      |   <Frame>
      |     <Id>Frame1</Id>
      |     <Value>
      |       <Name>F1</Name>
      |       <Origin>
      |         <Source>CenterOfMassFrame</Source>
      |         <FeatureName></FeatureName>
      |       </Origin>
      |       <PrimaryAxis>
      |         <DefinedDirection>+X</DefinedDirection>
      |         <Source>ReferenceFrame</Source>
      |         <SourceDirection>+Y</SourceDirection>
      |         <FeatureName></FeatureName>
      |       </PrimaryAxis>
      |       <SecondaryAxis>
      |         <DefinedDirection>+Z</DefinedDirection>
      |         <Source>ReferenceFrame</Source>
      |         <SourceDirection>+X</SourceDirection>
      |         <FeatureName></FeatureName>
      |       </SecondaryAxis>
      |     </Value>
      |   </Frame>
      | 
      | </Frames>
  RR_WheelAxisTransform2 : sm_lib/Frames and Transforms/Rigid Transform  RotationMethod=StandardAxis  FollAlignAxisA=+X  BaseAlignAxisA=+Y  FollAlignAxisB=+Y  BaseAlignAxisB=+Z  RotationStandardAxis=+X  RotationAngle=-90  RotationAngleUnits=deg  RotationArbitraryAxis=[0 0 1]  RotationSequenceAxes=FollowerAxes  RotationSequence=XYX  RotationSequenceAngles=[0 0 0]  RotationSequenceAnglesUnits=deg  RotationMatrix=[1 0 0;0 1 0;0 0 1]  Quaternion=[1 0 0 0]  TranslationMethod=Cartesian  TranslationCartesianOffset=[0 0 0]  TranslationCartesianOffsetUnits=m  TranslationStandardAxis=+Z  TranslationStandardOffset=0  TranslationStandardOffsetUnits=m  TranslationROffset=0  TranslationROffsetUnits=m  TranslationThetaOffset=0  TranslationThetaOffsetUnits=deg  TranslationZOffset=0  TranslationZOffsetUnits=m
  RR_ang_vel : nesl_utility/PS-Simulink Converter  PhysicalDomain=network_engine_domain  SubClassName=ps_output  LeftPortType=input  RightPortType=output  PseudoPeriodic=off  Frequencies=[]  VectorFormat=inherit  Unit=rad/s  AffineConversion=off
  ReplanStartXLog : ToWorkspace  VariableName=replanStartXLog  SaveFormat=Timeseries  SampleTime=-1
  ReplanStartYLog : ToWorkspace  VariableName=replanStartYLog  SaveFormat=Timeseries  SampleTime=-1
  RouteSwitch : Switch  Threshold=0.5  SaturateOnIntegerOverflow=off  InputSameDT=off
  RoverTireContact_FL : Subsystem
      settings: PortSchema="{\"entries\":[{\"content\":{\"sides\":[{\"content\":{\"connectorIds\":[\"Out3\",\"LConn1\"]},\"type\":\"ConnectorPlacement.EquallySpacedRectSide\",\"uuid\":\"0d23a9a3-abae-4569-82d6-ca0467ec27dd\"},{\"content\":{\"connectorIds\":[\"Out1\",\"Out2\",\"RConn1\"],\"side\":\"RIGHT\"},\"type\":\"ConnectorPlacement.EquallySpacedRectSide\",\"uuid\":\"e1624b92-fd2d-478b-925d-2a7f0ebb496f\"},{\"content\":{\"side\":\"TOP\"},\"type\":\"ConnectorPlacement.EquallySpacedRectSide\",\"uuid\":\"05d58ffd-b551-4868-a109-38149a8bb516\"}]},\"type\":\"ConnectorPlacement.EquallySpacedConnector\",\"uuid\":\"fe032146-0428-4b17-b698-d54db428c40e\"}],\"packageUris\":[\"http://schema.mathworks.com/mf0/Connector/R2020b\"],\"version\":\"1.0\"}"
  RoverTireContact_FR : Subsystem
      settings: PortSchema="{\"entries\":[{\"content\":{\"sides\":[{\"content\":{\"connectorIds\":[\"Out3\",\"LConn1\"]},\"type\":\"ConnectorPlacement.EquallySpacedRectSide\",\"uuid\":\"d5b10463-f999-4384-a17f-5a2cdcd8ba89\"},{\"content\":{\"connectorIds\":[\"Out1\",\"Out2\",\"RConn1\"],\"side\":\"RIGHT\"},\"type\":\"ConnectorPlacement.EquallySpacedRectSide\",\"uuid\":\"d75ede52-3ede-4525-9287-f42572d3129d\"},{\"content\":{\"side\":\"TOP\"},\"type\":\"ConnectorPlacement.EquallySpacedRectSide\",\"uuid\":\"b17b5dcd-0bea-4de0-b6ee-007afd2a7799\"}]},\"type\":\"ConnectorPlacement.EquallySpacedConnector\",\"uuid\":\"d3138c6b-eeeb-4420-872d-202e2a2d4879\"}],\"packageUris\":[\"http://schema.mathworks.com/mf0/Connector/R2020b\"],\"version\":\"1.0\"}"
  RoverTireContact_RL : Subsystem
      settings: PortSchema="{\"entries\":[{\"content\":{\"sides\":[{\"content\":{\"connectorIds\":[\"LConn1\",\"Out3\"]},\"type\":\"ConnectorPlacement.EquallySpacedRectSide\",\"uuid\":\"d5b10463-f999-4384-a17f-5a2cdcd8ba89\"},{\"content\":{\"connectorIds\":[\"Out1\",\"Out2\",\"RConn1\"],\"side\":\"RIGHT\"},\"type\":\"ConnectorPlacement.EquallySpacedRectSide\",\"uuid\":\"d75ede52-3ede-4525-9287-f42572d3129d\"},{\"content\":{\"side\":\"TOP\"},\"type\":\"ConnectorPlacement.EquallySpacedRectSide\",\"uuid\":\"b17b5dcd-0bea-4de0-b6ee-007afd2a7799\"},{\"content\":{\"side\":\"BOTTOM\"},\"type\":\"ConnectorPlacement.EquallySpacedRectSide\",\"uuid\":\"2e2ea952-2a2f-48e1-93dd-680b1958ebf5\"}]},\"type\":\"ConnectorPlacement.EquallySpacedConnector\",\"uuid\":\"d3138c6b-eeeb-4420-872d-202e2a2d4879\"}],\"packageUris\":[\"http://schema.mathworks.com/mf0/Connector/R2020b\"],\"version\":\"1.0\"}"
  RoverTireContact_RR : Subsystem
      settings: PortSchema="{\"entries\":[{\"content\":{\"sides\":[{\"content\":{\"connectorIds\":[\"Out3\",\"LConn1\"]},\"type\":\"ConnectorPlacement.EquallySpacedRectSide\",\"uuid\":\"d5b10463-f999-4384-a17f-5a2cdcd8ba89\"},{\"content\":{\"connectorIds\":[\"Out1\",\"Out2\",\"RConn1\"],\"side\":\"RIGHT\"},\"type\":\"ConnectorPlacement.EquallySpacedRectSide\",\"uuid\":\"d75ede52-3ede-4525-9287-f42572d3129d\"},{\"content\":{\"side\":\"TOP\"},\"type\":\"ConnectorPlacement.EquallySpacedRectSide\",\"uuid\":\"b17b5dcd-0bea-4de0-b6ee-007afd2a7799\"}]},\"type\":\"ConnectorPlacement.EquallySpacedConnector\",\"uuid\":\"d3138c6b-eeeb-4420-872d-202e2a2d4879\"}],\"packageUris\":[\"http://schema.mathworks.com/mf0/Connector/R2020b\"],\"version\":\"1.0\"}"
  Scope{,1..2,4..11,13..14} (13 alike) : Scope
      Scope settings: ActiveDisplayYMinimum=-399.28700335611506  ActiveDisplayYMaximum=646.10239319800826
      Scope1 settings: ActiveDisplayYMinimum=-0.97287290265374571  ActiveDisplayYMaximum=2.6837029972484139
      Scope10 settings: ActiveDisplayYMinimum=-69.490480255666242  ActiveDisplayYMaximum=85.047202917723055  DataLoggingVariableName=ScopeData11
      Scope11 settings: ActiveDisplayYMinimum=-27.107056427163915  ActiveDisplayYMaximum=31.136571068446493  DataLoggingVariableName=ScopeData12
      Scope13 settings: ActiveDisplayYMinimum=-2.4198479626678537  ActiveDisplayYMaximum=3.3579839981849071  DataLoggingVariableName=ScopeData14
      Scope14 settings: ActiveDisplayYMinimum=-2.2376009244028636  ActiveDisplayYMaximum=4.4509617992793071  DataLoggingVariableName=ScopeData15
      Scope2 settings: ActiveDisplayYMinimum=-161.14955439754061  ActiveDisplayYMaximum=932.66163232160477  DataLoggingVariableName=ScopeData2
      Scope4 settings: ActiveDisplayYMinimum=-19.791660434421718  ActiveDisplayYMaximum=19.629919241943707  DataLoggingVariableName=ScopeData4
      Scope5 settings: ActiveDisplayYMinimum=-224.64090504859431  ActiveDisplayYMaximum=148.94281283386556  DataLoggingVariableName=ScopeData5
      Scope6 settings: ActiveDisplayYMinimum=-149.86834533834616  ActiveDisplayYMaximum=127.65913059738848  DataLoggingVariableName=ScopeData7
      Scope7 settings: ActiveDisplayYMinimum=-81.715306101440618  ActiveDisplayYMaximum=136.71135648434415  DataLoggingVariableName=ScopeData8
      Scope8 settings: ActiveDisplayYMinimum=-81.715306101440618  ActiveDisplayYMaximum=136.71135648434415  DataLoggingVariableName=ScopeData9
      Scope9 settings: ActiveDisplayYMinimum=-109.81212441732507  ActiveDisplayYMaximum=168.96179779932069  DataLoggingVariableName=ScopeData10
  Scope12 : Scope  NumInputPorts=4
      settings: ActiveDisplayYMinimum=-1.8646695043634245  ActiveDisplayYMaximum=2.612385808037097  DataLoggingVariableName=ScopeData13
  Scope15 : Scope  NumInputPorts=7
      settings: ActiveDisplayYMinimum=-8.42239929091069  ActiveDisplayYMaximum=32.05094778821222  DataLoggingVariableName=ScopeData17
  Scope16 : Scope  NumInputPorts=4
      settings: ActiveDisplayYMinimum=-1  ActiveDisplayYMaximum=1  DataLoggingVariableName=ScopeData22
  Scope19 : Scope  NumInputPorts=3
      settings: ActiveDisplayYMinimum=-0.5075788039837974  ActiveDisplayYMaximum=4.7990166063050559  DataLoggingVariableName=ScopeData25
  Scope3 : Scope  NumInputPorts=2
      settings: ActiveDisplayYMinimum=-25.16119164032613  ActiveDisplayYMaximum=21.10271612930698  DataLoggingVariableName=ScopeData3
  SensorDetectionLog : ToWorkspace  VariableName=sensorDetectedLog  SaveFormat=Timeseries  SampleTime=-1
  Simulink-PS Converter{,1..3} (4 alike) : nesl_utility/Simulink-PS Converter  PhysicalDomain=network_engine_domain  SubClassName=ps_input  LeftPortType=input  RightPortType=output  PseudoPeriodic=off  Frequencies=[]  NoiseDistribution=none  NoiseParameters=[]  Unit=N*m  AffineConversion=off  FilteringAndDerivatives=provide  SimscapeFilterOrder=1  InputFilterTimeConstant=0.001  UdotUserProvided=0
  Simulink-PS Converter4 : nesl_utility/Simulink-PS Converter  PhysicalDomain=network_engine_domain  SubClassName=ps_input  LeftPortType=input  RightPortType=output  PseudoPeriodic=off  Frequencies=[]  NoiseDistribution=none  NoiseParameters=[]  Unit=rad  AffineConversion=off  FilteringAndDerivatives=filter  SimscapeFilterOrder=2  InputFilterTimeConstant=0.01  UdotUserProvided=0
  Simulink-PS Converter5 : nesl_utility/Simulink-PS Converter  PhysicalDomain=network_engine_domain  SubClassName=ps_input  LeftPortType=input  RightPortType=output  PseudoPeriodic=off  Frequencies=[]  NoiseDistribution=none  NoiseParameters=[]  Unit=rad  AffineConversion=off  FilteringAndDerivatives=filter  SimscapeFilterOrder=2  InputFilterTimeConstant=0.01  UdotUserProvided=0
  Solver Configuration : nesl_utility/Solver Configuration  PhysicalDomain=network_engine_domain  SubClassName=solver  LeftPortType=input  RightPortType=generic  Tones=[]  Harmonics=[]  SimulateNoise=off  Profile=off  UseLocalSampling=off  EnableSwitchedLinearOptims=on  FrequencyDomain=off  UseCCode=off  RelTol=0.001  AbsTol=1e-06  MinStep=1e-09  ToWorkspace=off  RevertToSquareIcSolve=off  NumHomotopyIterations=100  PhasorMode=off  PhasorModeNumHarmonics=1  ConsistencySolver=NEWTON_XTOL_AFTER_FTOL  CanonicalOrdering=UNORDERED  OptimizeIntermediates=UNOPTIMIZED  IndexReductionMethod=DerivativeReplacement  DoDC=off  ResidualTolerance=1e-09  ConsistencyTolSource=GLOBAL  ConsistencyAbsTol=0.001  ConsistencyRelTol=0.001  ConsistencyTolFactor=0.001  UseLocalSolver=off  LocalSolverChoice=NE_BACKWARD_EULER_ADVANCER  ResolveIndetEquations=on  FunctionEvalNumThread=1  LocalSolverSampleTime=0.001  DoFixedCost=off  MaxNonlinIter=3  MaxModeIter=2  ComputeImpulses=off  ImpulseIterations=2  LinearAlgebra=Sparse  LinearAlgebraNumThread=0  EquationFormulation=NE_TIME_EF  DelaysMemoryBudget=1024  AutomaticFiltering=on  FilteringTimeConstant=0.001  PartitionStorageMethod=AS_NEEDED  PartitionMemoryBudget=1024  PartitionMethod=FAST  MultibodyUseLocalSolver=off  MultibodyLocalSolverChoice=ODE1  MultibodyLocalSolverSampleTime=0.001
  Spatial Contact Force : sm_lib/Forces and Torques/Spatial Contact Force  SenseSeparationDistance=off  NormalForceType=SmoothSpringDamper  NormalStiffness=1e6  NormalStiffnessUnits=N/m  NormalDamping=1e3  NormalDampingUnits=N/(m/s)  NormalTransitionRegionWidth=1e-4  NormalTransitionRegionWidthUnits=m  FrictionType=SmoothStickSlip  CoefficientOfStaticFriction=0.5  CoefficientOfDynamicFriction=0.3  FrictionalCriticalVelocity=1e-3  FrictionalCriticalVelocityUnits=m/s  SenseContactSignal=on  SensePenetrationDepth=on  SenseNormalVelocity=off  SenseTangentialVelocity=off  SensingForceTorqueDirection=BaseOnFollower  SensingForceTorqueResolutionFrame=ContactFrame  SenseNormalForce=off  SenseNormalForceMagnitude=on  SenseNormalTorque=off  SenseFrictionalForce=off  SenseFrictionalForceMagnitude=off  SenseFrictionalTorque=off  SenseTotalForce=off  SenseTotalTorque=off  SenseContactBaseRotation=off  SenseContactBaseTranslation=off  SenseContactFollowerRotation=off  SenseContactFollowerTranslation=off  ZeroCrossDetectContactStartAndEnd=off
  Spatial Contact Force Obstacle2 : sm_lib/Forces and Torques/Spatial Contact Force  SenseSeparationDistance=off  NormalForceType=SmoothSpringDamper  NormalStiffness=1e6  NormalStiffnessUnits=N/m  NormalDamping=1e3  NormalDampingUnits=N/(m/s)  NormalTransitionRegionWidth=1e-4  NormalTransitionRegionWidthUnits=m  FrictionType=SmoothStickSlip  CoefficientOfStaticFriction=0.5  CoefficientOfDynamicFriction=0.3  FrictionalCriticalVelocity=1e-3  FrictionalCriticalVelocityUnits=m/s  SenseContactSignal=off  SensePenetrationDepth=off  SenseNormalVelocity=off  SenseTangentialVelocity=off  SensingForceTorqueDirection=BaseOnFollower  SensingForceTorqueResolutionFrame=ContactFrame  SenseNormalForce=off  SenseNormalForceMagnitude=off  SenseNormalTorque=off  SenseFrictionalForce=off  SenseFrictionalForceMagnitude=off  SenseFrictionalTorque=off  SenseTotalForce=off  SenseTotalTorque=off  SenseContactBaseRotation=off  SenseContactBaseTranslation=off  SenseContactFollowerRotation=off  SenseContactFollowerTranslation=off  ZeroCrossDetectContactStartAndEnd=off
  Spatial Contact Force Obstacle3 : sm_lib/Forces and Torques/Spatial Contact Force  SenseSeparationDistance=off  NormalForceType=SmoothSpringDamper  NormalStiffness=1e6  NormalStiffnessUnits=N/m  NormalDamping=1e3  NormalDampingUnits=N/(m/s)  NormalTransitionRegionWidth=1e-4  NormalTransitionRegionWidthUnits=m  FrictionType=SmoothStickSlip  CoefficientOfStaticFriction=0.5  CoefficientOfDynamicFriction=0.3  FrictionalCriticalVelocity=1e-3  FrictionalCriticalVelocityUnits=m/s  SenseContactSignal=off  SensePenetrationDepth=off  SenseNormalVelocity=off  SenseTangentialVelocity=off  SensingForceTorqueDirection=BaseOnFollower  SensingForceTorqueResolutionFrame=ContactFrame  SenseNormalForce=off  SenseNormalForceMagnitude=off  SenseNormalTorque=off  SenseFrictionalForce=off  SenseFrictionalForceMagnitude=off  SenseFrictionalTorque=off  SenseTotalForce=off  SenseTotalTorque=off  SenseContactBaseRotation=off  SenseContactBaseTranslation=off  SenseContactFollowerRotation=off  SenseContactFollowerTranslation=off  ZeroCrossDetectContactStartAndEnd=off
  Steering Revolute FL : sm_lib/Joints/Revolute Joint  JointMode=Normal  CompositeWrenchDir=FollowerOnBase  CompositeWrenchFrame=BaseFrame  SenseConstraintForce=off  SenseConstraintTorque=off  SenseTotalForce=off  SenseTotalTorque=off  PositionTargetSpecify=off  PositionTargetPriority=High  PositionTargetValue=0  PositionTargetValueUnits=deg  VelocityTargetSpecify=off  VelocityTargetPriority=High  VelocityTargetValue=0  VelocityTargetValueUnits=deg/s  EquilibriumPosition=0  EquilibriumPositionUnits=deg  SpringStiffness=0  SpringStiffnessUnits=N*m/deg  DampingCoefficient=0  DampingCoefficientUnits=N*m/(deg/s)  LowerLimitSpecify=off  LowerLimitBound=-90  LowerLimitBoundUnits=deg  LowerLimitStiffness=1e4  LowerLimitStiffnessUnits=N*m/deg  LowerLimitDamping=10  LowerLimitDampingUnits=N*m/(deg/s)  LowerLimitTransitionRegionWidth=0.1  LowerLimitTransitionRegionWidthUnits=deg  UpperLimitSpecify=off  UpperLimitBound=90  UpperLimitBoundUnits=deg  UpperLimitStiffness=1e4  UpperLimitStiffnessUnits=N*m/deg  UpperLimitDamping=10  UpperLimitDampingUnits=N*m/(deg/s)  UpperLimitTransitionRegionWidth=0.1  UpperLimitTransitionRegionWidthUnits=deg  TorqueActuationMode=ComputedTorque  MotionActuationMode=InputMotion  SensePosition=off  SenseVelocity=off  SenseAcceleration=off  SenseTorqueForce=off  SenseLowerLimitTorqueForce=off  SenseUpperLimitTorqueForce=off
  Steering Revolute FR : sm_lib/Joints/Revolute Joint  JointMode=Normal  CompositeWrenchDir=FollowerOnBase  CompositeWrenchFrame=BaseFrame  SenseConstraintForce=off  SenseConstraintTorque=off  SenseTotalForce=off  SenseTotalTorque=off  PositionTargetSpecify=off  PositionTargetPriority=High  PositionTargetValue=0  PositionTargetValueUnits=deg  VelocityTargetSpecify=off  VelocityTargetPriority=High  VelocityTargetValue=0  VelocityTargetValueUnits=deg/s  EquilibriumPosition=0  EquilibriumPositionUnits=deg  SpringStiffness=0  SpringStiffnessUnits=N*m/deg  DampingCoefficient=0  DampingCoefficientUnits=N*m/(deg/s)  LowerLimitSpecify=off  LowerLimitBound=-90  LowerLimitBoundUnits=deg  LowerLimitStiffness=1e4  LowerLimitStiffnessUnits=N*m/deg  LowerLimitDamping=10  LowerLimitDampingUnits=N*m/(deg/s)  LowerLimitTransitionRegionWidth=0.1  LowerLimitTransitionRegionWidthUnits=deg  UpperLimitSpecify=off  UpperLimitBound=90  UpperLimitBoundUnits=deg  UpperLimitStiffness=1e4  UpperLimitStiffnessUnits=N*m/deg  UpperLimitDamping=10  UpperLimitDampingUnits=N*m/(deg/s)  UpperLimitTransitionRegionWidth=0.1  UpperLimitTransitionRegionWidthUnits=deg  TorqueActuationMode=ComputedTorque  MotionActuationMode=InputMotion  SensePosition=off  SenseVelocity=off  SenseAcceleration=off  SenseTorqueForce=off  SenseLowerLimitTorqueForce=off  SenseUpperLimitTorqueForce=off
  Sum : Sum  Inputs=|+-
  Sum of Elements : Sum  Inputs=+
  Transfer Fcn : TransferFcn  Denominator=[0.15 1]
  Transform Sensor : sm_lib/Frames and Transforms/Transform Sensor  MeasurementFrame=World  RotationSequence=XYX  SenseAngle=off  SenseAxis=off  SenseQ=off  SenseR=off  SenseRotationSequence=off  SenseOmegaX=off  SenseOmegaY=off  SenseOmegaZ=off  SenseOmega=off  SenseQDot=off  SenseRDot=off  SenseRotationSequenceDot=off  SenseAlphaX=off  SenseAlphaY=off  SenseAlphaZ=off  SenseAlpha=off  SenseQDDot=off  SenseRDDot=off  SenseX=on  SenseY=off  SenseZ=off  SenseXYZ=off  SenseRad=off  SenseAzim=off  SenseDist=off  SenseInc=off  SenseXDot=on  SenseYDot=off  SenseZDot=off  SenseXYZDot=off  SenseRadDot=off  SenseAzimDot=off  SenseDistDot=off  SenseIncDot=off  SenseXDDot=off  SenseYDDot=off  SenseZDDot=off  SenseXYZDDot=off  SenseRadDDot=off  SenseAzimDDot=off  SenseDistDDot=off  SenseIncDDot=off
  Transform Sensor1 : sm_lib/Frames and Transforms/Transform Sensor  MeasurementFrame=World  RotationSequence=XYX  SenseAngle=off  SenseAxis=off  SenseQ=off  SenseR=off  SenseRotationSequence=off  SenseOmegaX=off  SenseOmegaY=off  SenseOmegaZ=off  SenseOmega=off  SenseQDot=off  SenseRDot=off  SenseRotationSequenceDot=off  SenseAlphaX=off  SenseAlphaY=off  SenseAlphaZ=off  SenseAlpha=off  SenseQDDot=off  SenseRDDot=off  SenseX=on  SenseY=on  SenseZ=on  SenseXYZ=off  SenseRad=off  SenseAzim=off  SenseDist=off  SenseInc=off  SenseXDot=off  SenseYDot=off  SenseZDot=off  SenseXYZDot=off  SenseRadDot=off  SenseAzimDot=off  SenseDistDot=off  SenseIncDot=off  SenseXDDot=off  SenseYDDot=off  SenseZDDot=off  SenseXYZDDot=off  SenseRadDDot=off  SenseAzimDDot=off  SenseDistDDot=off  SenseIncDDot=off
  Transform Sensor2 : sm_lib/Frames and Transforms/Transform Sensor  MeasurementFrame=World  RotationSequence=XYX  SenseAngle=off  SenseAxis=off  SenseQ=off  SenseR=off  SenseRotationSequence=off  SenseOmegaX=off  SenseOmegaY=off  SenseOmegaZ=off  SenseOmega=off  SenseQDot=off  SenseRDot=off  SenseRotationSequenceDot=off  SenseAlphaX=off  SenseAlphaY=off  SenseAlphaZ=off  SenseAlpha=off  SenseQDDot=off  SenseRDDot=off  SenseX=on  SenseY=on  SenseZ=on  SenseXYZ=off  SenseRad=off  SenseAzim=off  SenseDist=off  SenseInc=off  SenseXDot=off  SenseYDot=off  SenseZDot=off  SenseXYZDot=off  SenseRadDot=off  SenseAzimDot=off  SenseDistDot=off  SenseIncDot=off  SenseXDDot=off  SenseYDDot=off  SenseZDDot=off  SenseXYZDDot=off  SenseRadDDot=off  SenseAzimDDot=off  SenseDistDDot=off  SenseIncDDot=off
  WheelContactStatus : Mux
  WheelNormalLoads : Mux
  World Frame : sm_lib/Frames and Transforms/World Frame
  X : ToWorkspace  VariableName=mb_px  SaveFormat=Timeseries  SampleTime=-1
      settings: Decimation=20
  Y : ToWorkspace  VariableName=mb_py  SaveFormat=Timeseries  SampleTime=-1
      settings: Decimation=20
  goalX : Constant  Value=goalX
  goalY : Constant  Value=goalY
  velocity : nesl_utility/PS-Simulink Converter  PhysicalDomain=network_engine_domain  SubClassName=ps_output  LeftPortType=input  RightPortType=output  PseudoPeriodic=off  Frequencies=[]  VectorFormat=inherit  Unit=m/s  AffineConversion=off
  x : nesl_utility/PS-Simulink Converter  PhysicalDomain=network_engine_domain  SubClassName=ps_output  LeftPortType=input  RightPortType=output  PseudoPeriodic=off  Frequencies=[]  VectorFormat=inherit  Unit=m  AffineConversion=off
  x1 : nesl_utility/PS-Simulink Converter  PhysicalDomain=network_engine_domain  SubClassName=ps_output  LeftPortType=input  RightPortType=output  PseudoPeriodic=off  Frequencies=[]  VectorFormat=inherit  Unit=m  AffineConversion=off
  x2 : nesl_utility/PS-Simulink Converter  PhysicalDomain=network_engine_domain  SubClassName=ps_output  LeftPortType=input  RightPortType=output  PseudoPeriodic=off  Frequencies=[]  VectorFormat=inherit  Unit=m  AffineConversion=off
  y1 : nesl_utility/PS-Simulink Converter  PhysicalDomain=network_engine_domain  SubClassName=ps_output  LeftPortType=input  RightPortType=output  PseudoPeriodic=off  Frequencies=[]  VectorFormat=inherit  Unit=m  AffineConversion=off
  y2 : nesl_utility/PS-Simulink Converter  PhysicalDomain=network_engine_domain  SubClassName=ps_output  LeftPortType=input  RightPortType=output  PseudoPeriodic=off  Frequencies=[]  VectorFormat=inherit  Unit=m  AffineConversion=off
  z1 : nesl_utility/PS-Simulink Converter  PhysicalDomain=network_engine_domain  SubClassName=ps_output  LeftPortType=input  RightPortType=output  PseudoPeriodic=off  Frequencies=[]  VectorFormat=inherit  Unit=m  AffineConversion=off
  z2 : nesl_utility/PS-Simulink Converter  PhysicalDomain=network_engine_domain  SubClassName=ps_output  LeftPortType=input  RightPortType=output  PseudoPeriodic=off  Frequencies=[]  VectorFormat=inherit  Unit=m  AffineConversion=off
  wires:
  RoverTireContact_RR/1(Fz) -> WheelNormalLoads/1
  RoverTireContact_RL/1(Fz) -> WheelNormalLoads/2
  RoverTireContact_FL/1(Fz) -> WheelNormalLoads/3
  RoverTireContact_FR/1(Fz) -> WheelNormalLoads/4
  RoverTireContact_RR/2(Contact) -> WheelContactStatus/1
  RoverTireContact_RL/2(Contact) -> WheelContactStatus/2
  RoverTireContact_FL/2(Contact) -> WheelContactStatus/3
  RoverTireContact_FR/2(Contact) -> WheelContactStatus/4
  WheelNormalLoads/1 -> Sum of Elements/1, Scope/1
  WheelContactStatus/1 -> Scope1/1
  Sum of Elements/1 -> Scope2/1  "TotalNormalForce"
  x/1 -> Scope3/1
  velocity/1 -> Scope3/2
  FL_ang_vel/1 -> Scope4/1
  RoverTireContact_FL/3(Fx) -> Scope5/1
  FR_ang_vel/1 -> Scope6/1
  RoverTireContact_FR/3(Fx) -> Scope7/1
  RoverTireContact_RL/3(Fx) -> Scope8/1
  RoverTireContact_RR/3(Fx) -> Scope9/1
  RL_ang_vel/1 -> Scope10/1
  RR_ang_vel/1 -> Scope11/1
  Gain/1 -> Scope12/2, Simulink-PS Converter3/1  "Drive Torque RR"
  Gain1/1 -> Simulink-PS Converter2/1, Scope12/4  "Drive Torque RL"
  Gain3/1 -> Scope12/3, Simulink-PS Converter/1  "Drive Torque FL"
  Gain2/1 -> Scope12/1, Simulink-PS Converter1/1  "Drive Torque FR"
  PID Controller/1 -> Gain2/1, Gain/1, Gain1/1, Gain3/1  "Drive Torque"
  PurePursuitController/2(speedRef) -> GoalStopLogic/3(vRef)
  Sum/1 -> PID Controller/1
  PS-Simulink Converter/1 -> Scope13/1  "Feedback velocity to PI"
  PS-Simulink Converter1/1 -> GoalStopLogic/1(x), OnlineReplanManager/1(x), ObstacleSensorLogic/1(x), X/1, PurePursuitController/1(x), Scope15/1  "px"
  PS-Simulink Converter3/1 -> Y/1, GoalStopLogic/2(y), OnlineReplanManager/2(y), ObstacleSensorLogic/2(y), PurePursuitController/2(y), Scope15/4  "py"
  PS-Simulink Converter2/1 -> LongitudinalVelocity/2(vy), Scope15/2  "vy"
  PS-Simulink Converter5/1 -> Scope15/3  "pz"
  PS-Simulink Converter4/1 -> Demux/1, Scope15/5  "Q"
  PS-Simulink Converter6/1 -> Scope16/2, LongitudinalVelocity/1(vx), Scope15/7  "vx"
  PS-Simulink Converter7/1 -> Scope15/6  "wz"
  PS-Simulink Converter9/1 -> RR Prismatic joint/2  "prismatic position"
  PS-Simulink Converter8/1 -> RR Prismatic joint/1  "prismatic velocity"
  PS-Simulink Converter11/1 -> RL Prismatic joint/2  "prismatic position"
  PS-Simulink Converter10/1 -> RL Prismatic joint/1  "prismatic velocity"
  PS-Simulink Converter13/1 -> FL Prismatic joint/2  "prismatic position"
  PS-Simulink Converter12/1 -> FL Prismatic joint/1  "prismatic velocity"
  PS-Simulink Converter15/1 -> FR Prismatic joint/1  "prismatic position"
  PS-Simulink Converter14/1 -> FR Prismatic joint/2  "prismatic velocity"
  AckermannSteering/2(deltaFR) -> Probe_ToWorkspace_deltaFRProbe/1, Simulink-PS Converter4/1, Scope16/4
  AckermannSteering/1(deltaFL) -> Scope16/3, Simulink-PS Converter5/1, Probe_ToWorkspace_deltaFLProbe/1
  Demux/1 -> PurePursuitController/3(q0), LongitudinalVelocity/3(q0), ObstacleSensorLogic/3(q0)
  Demux/4 -> PurePursuitController/6(q3), ObstacleSensorLogic/6(q3), LongitudinalVelocity/6(q3)
  Demux/2 -> PurePursuitController/4(q1), LongitudinalVelocity/4(q1), ObstacleSensorLogic/4(q1)
  Demux/3 -> PurePursuitController/5(q2), ObstacleSensorLogic/5(q2), LongitudinalVelocity/5(q2)
  PurePursuitController/1(steerCmd) -> Probe_ToWorkspace_steerCmdProbe/1, Transfer Fcn/1, Scope16/1  "steerCmd"
  GoalStopLogic/1(vCmd) -> Sum/1
  LongitudinalVelocity/1(vLong) -> Sum/2, Scope14/1
  Transfer Fcn/1 -> AckermannSteering/1(delta), Probe_ToWorkspace_deltaFilteredProbe/1
  goalX/1 -> OnlineReplanManager/4(goalX), GoalStopLogic/4(goalX)
  goalY/1 -> OnlineReplanManager/5(goalY), GoalStopLogic/5(goalY)
  ObstacleSensorLogic/1(detected) -> SensorDetectionLog/1  "sensorDetected"
  PathWaypoints/1 -> RouteSwitch/3
  RouteSwitch/1 -> PurePursuitController/7(wp), Probe_ToWorkspace_routeInputProbe/1
  ObstacleX/1 -> DynamicObstacleEnvironment/2(knownXs)
  ObstacleY/1 -> DynamicObstacleEnvironment/3(knownYs)
  OnlineReplanManager/1(route) -> RouteSwitch/1
  OnlineReplanManager/4(replanStartX) -> ReplanStartXLog/1
  OnlineReplanManager/5(replanStartY) -> ReplanStartYLog/1
  ObstacleSensorLogic/3(detectedX) -> OnlineReplanManager/6(detectedX)
  ObstacleSensorLogic/4(detectedY) -> OnlineReplanManager/7(detectedY)
  ObstacleSensorLogic/2(newDetection) -> OnlineReplanManager/3(newDetection)
  OnlineReplanManager/3(replanEvent) -> OnlineReplanEventLog/1
  OnlineReplanManager/2(routeReady) -> RouteSwitch/2
  Clock/1 -> DynamicObstacleEnvironment/1(t)
  Obstacle3X/1 -> DynamicObstacleEnvironment/4(obstacle3X)
  Obstacle3Y/1 -> DynamicObstacleEnvironment/5(obstacle3Y)
  ObstacleSpawnTime/1 -> DynamicObstacleEnvironment/6(spawnTime)
  DynamicObstacleEnvironment/1(environmentXs) -> ObstacleSensorLogic/7(environmentXs)
  DynamicObstacleEnvironment/2(environmentYs) -> ObstacleSensorLogic/8(environmentYs)
  PS-Simulink Converter18/1 -> Scope19/1  "CON"
  PS-Simulink Converter17/1 -> Scope19/2  "pen"
  PS-Simulink Converter16/1 -> Scope19/3  "fnm"
  Obstacle2SpawnModeStep/1 -> Obstacle2ModeConverter/1
  Obstacle3SpawnModeStep/1 -> Obstacle3ModeConverter/1
  x1/1 -> FR_Revolute Sensor/1
  y1/1 -> FR_Revolute Sensor/2
  z1/1 -> FR_Revolute Sensor/3
  y2/1 -> FL_Revolute Sensor/2
  x2/1 -> FL_Revolute Sensor/1
  z2/1 -> FL_Revolute Sensor/3
  connections:
  World Frame/RConn1 -- Obstacle2Placement/LConn1 -- Obstacle3Placement/LConn1 -- 6-DOF Joint/LConn1 -- Solver Configuration/RConn1 -- Transform Sensor2/LConn1 -- Transform Sensor1/LConn1 -- Transform Sensor/LConn1 -- Mechanism Configuration/RConn1 -- Grid Surface/LConn1 -- Obstacle1Placement/LConn1
  6-DOF Joint/RConn1 -- Transform Sensor/RConn1 -- FR_RigidTransform/LConn1 -- FL_RigidTransform/LConn1 -- Chassis/LConn1 -- RR_RigidTransform/LConn1 -- RL_RigidTransform/LConn1
  FR_Revolute/RConn1 -- Transform Sensor1/RConn1 -- RoverTireContact_FR/RConn1 -- FR_Wheel/LConn1
  RR_Revolute/LConn1 -- RR_WheelAxisTransform2/RConn1
  RR_Revolute/RConn1 -- RR_Wheel/LConn1 -- RoverTireContact_RR/RConn1
  RL_Revolute/LConn1 -- RL_WheelAxisTransform/RConn1
  RL_Revolute/RConn1 -- RL_Wheel/LConn1 -- RoverTireContact_RL/RConn1
  FL_Revolute/RConn1 -- RoverTireContact_FL/RConn1 -- Transform Sensor2/RConn1 -- FL_Wheel/LConn1
  Grid Surface/RConn1 -- RoverTireContact_RR/LConn1 -- RoverTireContact_RL/LConn1 -- RoverTireContact_FL/LConn1 -- RoverTireContact_FR/LConn1
  FL_RigidTransform/RConn1 -- Steering Revolute FL/LConn1
  Prismatic Joint/RConn1 -- FL_WheelAxisTransform/LConn1
  FL_WheelAxisTransform/RConn1 -- FL_Revolute/LConn1
  FR_WheelAxisTransform/LConn1 -- Prismatic Joint1/RConn1
  Prismatic Joint2/LConn1 -- RL_RigidTransform/RConn1
  RL_WheelAxisTransform/LConn1 -- Prismatic Joint2/RConn1
  Prismatic Joint3/LConn1 -- RR_RigidTransform/RConn1
  RR_WheelAxisTransform2/LConn1 -- Prismatic Joint3/RConn1
  x/LConn1 -- Transform Sensor/RConn2
  velocity/LConn1 -- Transform Sensor/RConn3
  FL_Revolute/LConn2 -- Simulink-PS Converter/RConn1
  FL_Revolute/RConn2 -- FL_ang_vel/LConn1
  FR_Revolute/LConn1 -- FR_WheelAxisTransform/RConn1
  Simulink-PS Converter1/RConn1 -- FR_Revolute/LConn2
  FR_ang_vel/LConn1 -- FR_Revolute/RConn2
  Simulink-PS Converter2/RConn1 -- RL_Revolute/LConn2
  RL_ang_vel/LConn1 -- RL_Revolute/RConn2
  Simulink-PS Converter3/RConn1 -- RR_Revolute/LConn2
  RR_Revolute/RConn2 -- RR_ang_vel/LConn1
  6-DOF Joint/RConn3 -- PS-Simulink Converter/LConn1 -- PS-Simulink Converter6/LConn1
  6-DOF Joint/RConn2 -- PS-Simulink Converter1/LConn1
  PS-Simulink Converter3/LConn1 -- 6-DOF Joint/RConn4
  PS-Simulink Converter2/LConn1 -- 6-DOF Joint/RConn5
  6-DOF Joint/RConn6 -- PS-Simulink Converter5/LConn1
  6-DOF Joint/RConn7 -- PS-Simulink Converter4/LConn1
  6-DOF Joint/RConn8 -- PS-Simulink Converter7/LConn1
  Prismatic Joint3/RConn2 -- PS-Simulink Converter9/LConn1
  Prismatic Joint3/RConn3 -- PS-Simulink Converter8/LConn1
  PS-Simulink Converter10/LConn1 -- Prismatic Joint2/RConn3
  PS-Simulink Converter11/LConn1 -- Prismatic Joint2/RConn2
  Prismatic Joint/RConn2 -- PS-Simulink Converter13/LConn1
  Prismatic Joint/RConn3 -- PS-Simulink Converter12/LConn1
  PS-Simulink Converter15/LConn1 -- Prismatic Joint1/RConn2
  PS-Simulink Converter14/LConn1 -- Prismatic Joint1/RConn3
  Steering Revolute FL/RConn1 -- Prismatic Joint/LConn1
  FR_RigidTransform/RConn1 -- Steering Revolute FR/LConn1
  Steering Revolute FR/RConn1 -- Prismatic Joint1/LConn1
  Simulink-PS Converter4/RConn1 -- Steering Revolute FR/LConn2
  Simulink-PS Converter5/RConn1 -- Steering Revolute FL/LConn2
  Spatial Contact Force/LConn1 -- Spatial Contact Force Obstacle3/LConn1 -- Spatial Contact Force Obstacle2/LConn1 -- Chassis/RConn1
  Spatial Contact Force/RConn1 -- PhysicalObstacle1/LConn1
  Obstacle1Placement/RConn1 -- PhysicalObstacle1/RConn1
  Spatial Contact Force/RConn2 -- PS-Simulink Converter18/LConn1
  Spatial Contact Force/RConn3 -- PS-Simulink Converter17/LConn1
  Spatial Contact Force/RConn4 -- PS-Simulink Converter16/LConn1
  Spatial Contact Force Obstacle2/RConn1 -- PhysicalObstacle2/LConn1
  Obstacle2Placement/RConn1 -- Obstacle2SpawnJoint/LConn1
  Obstacle2SpawnJoint/RConn1 -- PhysicalObstacle2/RConn1
  Obstacle2ModeConverter/RConn1 -- Obstacle2SpawnJoint/LConn2
  Spatial Contact Force Obstacle3/RConn1 -- PhysicalObstacle3/LConn1
  Obstacle3Placement/RConn1 -- Obstacle3SpawnJoint/LConn1
  Obstacle3SpawnJoint/RConn1 -- PhysicalObstacle3/RConn1
  Obstacle3ModeConverter/RConn1 -- Obstacle3SpawnJoint/LConn2
  x1/LConn1 -- Transform Sensor1/RConn2
  Transform Sensor1/RConn3 -- y1/LConn1
  z1/LConn1 -- Transform Sensor1/RConn4
  Transform Sensor2/RConn3 -- y2/LConn1
  z2/LConn1 -- Transform Sensor2/RConn4
  x2/LConn1 -- Transform Sensor2/RConn2
